simulink model "PV4x4_sweep_grp"  (R2025b)
(part 3 of 3)

  D_41_1 : ee_lib/Semiconductors & Converters/Diode  ModelType=ee.enum.diode.modelType.pwl  TableType=ee.enum.diode.tableType.IfMat  IfMat=[.07, .12, .19, 1.75, 4.24, 7.32, 11.2; .16, .3, .72, 2.14, 5.02, 8.35, 13.12] A  VfMat=[.9, 1.15, 1.25, 1.5, 1.75, 2.17, 2.6, 2.85; .58, .68, .75, 1.1, 1.38, 1.77, 2.27, 2.7] V  TjVec=[25, 125] degC  VfVec=[.5, .7, .9, 1.3, 1.7, 2.1, 2.5] V  IfVec=[.1, .2, .5, 1, 2, 4, 7, 10] A  IrMat=[1e-06, 2e-06, 5e-06, 1e-05, 2.5e-05, 5e-05, .0001; 2e-06, 5e-06, 1e-05, 4e-05, 8e-05, .0002, .0005] A  VrMat=[10, 100, 200, 250, 300, 325, 350; 10, 70, 160, 220, 270, 300, 320] V  VrVec=[10, 20, 40, 50, 70, 80, 100] V  IrVec=[1e-06, 2e-06, 5e-06, 1e-05, 2e-05, 5e-05, .0001] A  Vf=byp_Vf V  Ron=byp_Ron Ohm  Goff=byp_Goff S  prmExp=ee.enum.diode.expParam.useTwo  I12=[.0137, .545] A  V12=[.6, .7] V  RS=0 Ohm  Tmeas=298.15 K  IS=1e-12 A  ec=1  I1=0.0137 A  V1=0.6 V  N_series=1  N_parallel=1  ZenerEnable=false  Rz=0.3 Ohm  BV=inf V  C_param=ee.enum.diode.capParam.fixed  CJ=0 pF  CJ0=5 pF  Vvec=[.1, 10, 100] V  Cvec=[3.5, 1, .4] pF  VJ=1 V  Mgrad=0.5  FC=0.5  Q_param=ee.enum.diode.recoveryParam.off  iRM=-7.15 A  iF=4 A  didt=-750 A/us  trr_factor=3  trr=115 ns  Qrr=150 nA*s  Vr=-600 V  Ls=150 nH  Erec=0.03 J  TT=50 ns  tau=100 ns  T_param=ee.enum.diode.temperatureParam.off  Tdevice=298.15 K  I1_T2=0.245 A  V1_T2=0.5 V  IS_T2=1.25e-7 A  Tmeas2=125 degC  XTI_param=ee.enum.diode.xtiParam.pn  XTI=3  EG_param=ee.enum.diode.egapParam.material_si  EG=1.11 eV  dBVdT=0 V/K  enable_fault_input=simscape.enum.onoff.off  i_specify=off  i_priority=None  i=0 A  i_nominal_specify=off  i_nominal_value=1  i_nominal_unit=A  v_specify=off  v_priority=None  v=0 V  v_nominal_specify=off  v_nominal_value=1  v_nominal_unit=V  v_capacitor_specify=off  v_capacitor_priority=None  v_capacitor=0 V  v_capacitor_nominal_specify=off  v_capacitor_nominal_value=1  v_capacitor_nominal_unit=V  Qj_specify=off  Qj_priority=High  Qj=0 C  Qj_nominal_specify=off  Qj_nominal_value=1  Qj_nominal_unit=C  i_diode_specify=off  i_diode_priority=None  i_diode=0 A  i_diode_nominal_specify=off  i_diode_nominal_value=1  i_diode_nominal_unit=A  v_diode_specify=off  v_diode_priority=None  v_diode=0 V  v_diode_nominal_specify=off  v_diode_nominal_value=1  v_diode_nominal_unit=V  i_capacitor_specify=off  i_capacitor_priority=None  i_capacitor=0 A  i_capacitor_nominal_specify=off  i_capacitor_nominal_value=1  i_capacitor_nominal_unit=A  power_dissipated_specify=off  power_dissipated_priority=None  power_dissipated=0 W  power_dissipated_nominal_specify=off  power_dissipated_nominal_value=1  power_dissipated_nominal_unit=W  fidelity_level=ee.enum.diode.fidelity.includeChargeDyn  rec_loss_model=ee.enum.diode.reverseRecoveryModel.fixed  ErecVal=0 J  scaleWithIandV=true  ErecMat=zeros(2, 3) J  TjrecVec=[298.15, 398.15] K  IfrecVec=[.1, 1, 10] A  IrecVal=10 A  VrecVal=10 V  tFilter=1 / 1000 / 100 s  thermal_network_parameterization=ee.enum.thermalNetworkTopology.junctionCase  Rth=[0, 10] K/W  Rth_Cauer=[1, 3, 10] K/W  Rth_Foster=[.08, .14, .22, .16] K/W  thermal_mass_parameterization=ee.enum.thermalNetwork.timeconstant  thermal_mass=[0, 1] J/K  thermal_mass_Cauer=[.1, .3, 1] J/K  thermal_mass_Foster=[.001, .005, .05, .5] J/K  thermal_time_constant=[0, 10] s  thermal_time_constant_Cauer=[1, 3, 10] s  thermal_time_constant_Foster=[7e-05, .0007, .01, .08] s  thermal_mass_initial_temperatures=[25, 25] degC  thermal_mass_initial_temperatures_Cauer=[25, 25, 25] degC  junction_thermal_mass=0.01 J/K  Tvec_initial_Foster=[25, 25, 25, 25] degC  no_thermal_network=0  junction_temperature_specify=off  junction_temperature_priority=None  junction_temperature=25 degC  junction_temperature_nominal_specify=off  junction_temperature_nominal_value=1  junction_temperature_nominal_unit=degC
  D_41_2 : ee_lib/Semiconductors & Converters/Diode  ModelType=ee.enum.diode.modelType.pwl  TableType=ee.enum.diode.tableType.IfMat  IfMat=[.07, .12, .19, 1.75, 4.24, 7.32, 11.2; .16, .3, .72, 2.14, 5.02, 8.35, 13.12] A  VfMat=[.9, 1.15, 1.25, 1.5, 1.75, 2.17, 2.6, 2.85; .58, .68, .75, 1.1, 1.38, 1.77, 2.27, 2.7] V  TjVec=[25, 125] degC  VfVec=[.5, .7, .9, 1.3, 1.7, 2.1, 2.5] V  IfVec=[.1, .2, .5, 1, 2, 4, 7, 10] A  IrMat=[1e-06, 2e-06, 5e-06, 1e-05, 2.5e-05, 5e-05, .0001; 2e-06, 5e-06, 1e-05, 4e-05, 8e-05, .0002, .0005] A  VrMat=[10, 100, 200, 250, 300, 325, 350; 10, 70, 160, 220, 270, 300, 320] V  VrVec=[10, 20, 40, 50, 70, 80, 100] V  IrVec=[1e-06, 2e-06, 5e-06, 1e-05, 2e-05, 5e-05, .0001] A  Vf=byp_Vf V  Ron=byp_Ron Ohm  Goff=byp_Goff S  prmExp=ee.enum.diode.expParam.useTwo  I12=[.0137, .545] A  V12=[.6, .7] V  RS=0 Ohm  Tmeas=298.15 K  IS=1e-12 A  ec=1  I1=0.0137 A  V1=0.6 V  N_series=1  N_parallel=1  ZenerEnable=false  Rz=0.3 Ohm  BV=inf V  C_param=ee.enum.diode.capParam.fixed  CJ=0 pF  CJ0=5 pF  Vvec=[.1, 10, 100] V  Cvec=[3.5, 1, .4] pF  VJ=1 V  Mgrad=0.5  FC=0.5  Q_param=ee.enum.diode.recoveryParam.off  iRM=-7.15 A  iF=4 A  didt=-750 A/us  trr_factor=3  trr=115 ns  Qrr=150 nA*s  Vr=-600 V  Ls=150 nH  Erec=0.03 J  TT=50 ns  tau=100 ns  T_param=ee.enum.diode.temperatureParam.off  Tdevice=298.15 K  I1_T2=0.245 A  V1_T2=0.5 V  IS_T2=1.25e-7 A  Tmeas2=125 degC  XTI_param=ee.enum.diode.xtiParam.pn  XTI=3  EG_param=ee.enum.diode.egapParam.material_si  EG=1.11 eV  dBVdT=0 V/K  enable_fault_input=simscape.enum.onoff.off  i_specify=off  i_priority=None  i=0 A  i_nominal_specify=off  i_nominal_value=1  i_nominal_unit=A  v_specify=off  v_priority=None  v=0 V  v_nominal_specify=off  v_nominal_value=1  v_nominal_unit=V  v_capacitor_specify=off  v_capacitor_priority=None  v_capacitor=0 V  v_capacitor_nominal_specify=off  v_capacitor_nominal_value=1  v_capacitor_nominal_unit=V  Qj_specify=off  Qj_priority=High  Qj=0 C  Qj_nominal_specify=off  Qj_nominal_value=1  Qj_nominal_unit=C  i_diode_specify=off  i_diode_priority=None  i_diode=0 A  i_diode_nominal_specify=off  i_diode_nominal_value=1  i_diode_nominal_unit=A  v_diode_specify=off  v_diode_priority=None  v_diode=0 V  v_diode_nominal_specify=off  v_diode_nominal_value=1  v_diode_nominal_unit=V  i_capacitor_specify=off  i_capacitor_priority=None  i_capacitor=0 A  i_capacitor_nominal_specify=off  i_capacitor_nominal_value=1  i_capacitor_nominal_unit=A  power_dissipated_specify=off  power_dissipated_priority=None  power_dissipated=0 W  power_dissipated_nominal_specify=off  power_dissipated_nominal_value=1  power_dissipated_nominal_unit=W  fidelity_level=ee.enum.diode.fidelity.includeChargeDyn  rec_loss_model=ee.enum.diode.reverseRecoveryModel.fixed  ErecVal=0 J  scaleWithIandV=true  ErecMat=zeros(2, 3) J  TjrecVec=[298.15, 398.15] K  IfrecVec=[.1, 1, 10] A  IrecVal=10 A  VrecVal=10 V  tFilter=1 / 1000 / 100 s  thermal_network_parameterization=ee.enum.thermalNetworkTopology.junctionCase  Rth=[0, 10] K/W  Rth_Cauer=[1, 3, 10] K/W  Rth_Foster=[.08, .14, .22, .16] K/W  thermal_mass_parameterization=ee.enum.thermalNetwork.timeconstant  thermal_mass=[0, 1] J/K  thermal_mass_Cauer=[.1, .3, 1] J/K  thermal_mass_Foster=[.001, .005, .05, .5] J/K  thermal_time_constant=[0, 10] s  thermal_time_constant_Cauer=[1, 3, 10] s  thermal_time_constant_Foster=[7e-05, .0007, .01, .08] s  thermal_mass_initial_temperatures=[25, 25] degC  thermal_mass_initial_temperatures_Cauer=[25, 25, 25] degC  junction_thermal_mass=0.01 J/K  Tvec_initial_Foster=[25, 25, 25, 25] degC  no_thermal_network=0  junction_temperature_specify=off  junction_temperature_priority=None  junction_temperature=25 degC  junction_temperature_nominal_specify=off  junction_temperature_nominal_value=1  junction_temperature_nominal_unit=degC
  D_41_3 : ee_lib/Semiconductors & Converters/Diode  ModelType=ee.enum.diode.modelType.pwl  TableType=ee.enum.diode.tableType.IfMat  IfMat=[.07, .12, .19, 1.75, 4.24, 7.32, 11.2; .16, .3, .72, 2.14, 5.02, 8.35, 13.12] A  VfMat=[.9, 1.15, 1.25, 1.5, 1.75, 2.17, 2.6, 2.85; .58, .68, .75, 1.1, 1.38, 1.77, 2.27, 2.7] V  TjVec=[25, 125] degC  VfVec=[.5, .7, .9, 1.3, 1.7, 2.1, 2.5] V  IfVec=[.1, .2, .5, 1, 2, 4, 7, 10] A  IrMat=[1e-06, 2e-06, 5e-06, 1e-05, 2.5e-05, 5e-05, .0001; 2e-06, 5e-06, 1e-05, 4e-05, 8e-05, .0002, .0005] A  VrMat=[10, 100, 200, 250, 300, 325, 350; 10, 70, 160, 220, 270, 300, 320] V  VrVec=[10, 20, 40, 50, 70, 80, 100] V  IrVec=[1e-06, 2e-06, 5e-06, 1e-05, 2e-05, 5e-05, .0001] A  Vf=byp_Vf V  Ron=byp_Ron Ohm  Goff=byp_Goff S  prmExp=ee.enum.diode.expParam.useTwo  I12=[.0137, .545] A  V12=[.6, .7] V  RS=0 Ohm  Tmeas=298.15 K  IS=1e-12 A  ec=1  I1=0.0137 A  V1=0.6 V  N_series=1  N_parallel=1  ZenerEnable=false  Rz=0.3 Ohm  BV=inf V  C_param=ee.enum.diode.capParam.fixed  CJ=0 pF  CJ0=5 pF  Vvec=[.1, 10, 100] V  Cvec=[3.5, 1, .4] pF  VJ=1 V  Mgrad=0.5  FC=0.5  Q_param=ee.enum.diode.recoveryParam.off  iRM=-7.15 A  iF=4 A  didt=-750 A/us  trr_factor=3  trr=115 ns  Qrr=150 nA*s  Vr=-600 V  Ls=150 nH  Erec=0.03 J  TT=50 ns  tau=100 ns  T_param=ee.enum.diode.temperatureParam.off  Tdevice=298.15 K  I1_T2=0.245 A  V1_T2=0.5 V  IS_T2=1.25e-7 A  Tmeas2=125 degC  XTI_param=ee.enum.diode.xtiParam.pn  XTI=3  EG_param=ee.enum.diode.egapParam.material_si  EG=1.11 eV  dBVdT=0 V/K  enable_fault_input=simscape.enum.onoff.off  i_specify=off  i_priority=None  i=0 A  i_nominal_specify=off  i_nominal_value=1  i_nominal_unit=A  v_specify=off  v_priority=None  v=0 V  v_nominal_specify=off  v_nominal_value=1  v_nominal_unit=V  v_capacitor_specify=off  v_capacitor_priority=None  v_capacitor=0 V  v_capacitor_nominal_specify=off  v_capacitor_nominal_value=1  v_capacitor_nominal_unit=V  Qj_specify=off  Qj_priority=High  Qj=0 C  Qj_nominal_specify=off  Qj_nominal_value=1  Qj_nominal_unit=C  i_diode_specify=off  i_diode_priority=None  i_diode=0 A  i_diode_nominal_specify=off  i_diode_nominal_value=1  i_diode_nominal_unit=A  v_diode_specify=off  v_diode_priority=None  v_diode=0 V  v_diode_nominal_specify=off  v_diode_nominal_value=1  v_diode_nominal_unit=V  i_capacitor_specify=off  i_capacitor_priority=None  i_capacitor=0 A  i_capacitor_nominal_specify=off  i_capacitor_nominal_value=1  i_capacitor_nominal_unit=A  power_dissipated_specify=off  power_dissipated_priority=None  power_dissipated=0 W  power_dissipated_nominal_specify=off  power_dissipated_nominal_value=1  power_dissipated_nominal_unit=W  fidelity_level=ee.enum.diode.fidelity.includeChargeDyn  rec_loss_model=ee.enum.diode.reverseRecoveryModel.fixed  ErecVal=0 J  scaleWithIandV=true  ErecMat=zeros(2, 3) J  TjrecVec=[298.15, 398.15] K  IfrecVec=[.1, 1, 10] A  IrecVal=10 A  VrecVal=10 V  tFilter=1 / 1000 / 100 s  thermal_network_parameterization=ee.enum.thermalNetworkTopology.junctionCase  Rth=[0, 10] K/W  Rth_Cauer=[1, 3, 10] K/W  Rth_Foster=[.08, .14, .22, .16] K/W  thermal_mass_parameterization=ee.enum.thermalNetwork.timeconstant  thermal_mass=[0, 1] J/K  thermal_mass_Cauer=[.1, .3, 1] J/K  thermal_mass_Foster=[.001, .005, .05, .5] J/K  thermal_time_constant=[0, 10] s  thermal_time_constant_Cauer=[1, 3, 10] s  thermal_time_constant_Foster=[7e-05, .0007, .01, .08] s  thermal_mass_initial_temperatures=[25, 25] degC  thermal_mass_initial_temperatures_Cauer=[25, 25, 25] degC  junction_thermal_mass=0.01 J/K  Tvec_initial_Foster=[25, 25, 25, 25] degC  no_thermal_network=0  junction_temperature_specify=off  junction_temperature_priority=None  junction_temperature=25 degC  junction_temperature_nominal_specify=off  junction_temperature_nominal_value=1  junction_temperature_nominal_unit=degC
  D_42_1 : ee_lib/Semiconductors & Converters/Diode  ModelType=ee.enum.diode.modelType.pwl  TableType=ee.enum.diode.tableType.IfMat  IfMat=[.07, .12, .19, 1.75, 4.24, 7.32, 11.2; .16, .3, .72, 2.14, 5.02, 8.35, 13.12] A  VfMat=[.9, 1.15, 1.25, 1.5, 1.75, 2.17, 2.6, 2.85; .58, .68, .75, 1.1, 1.38, 1.77, 2.27, 2.7] V  TjVec=[25, 125] degC  VfVec=[.5, .7, .9, 1.3, 1.7, 2.1, 2.5] V  IfVec=[.1, .2, .5, 1, 2, 4, 7, 10] A  IrMat=[1e-06, 2e-06, 5e-06, 1e-05, 2.5e-05, 5e-05, .0001; 2e-06, 5e-06, 1e-05, 4e-05, 8e-05, .0002, .0005] A  VrMat=[10, 100, 200, 250, 300, 325, 350; 10, 70, 160, 220, 270, 300, 320] V  VrVec=[10, 20, 40, 50, 70, 80, 100] V  IrVec=[1e-06, 2e-06, 5e-06, 1e-05, 2e-05, 5e-05, .0001] A  Vf=byp_Vf V  Ron=byp_Ron Ohm  Goff=byp_Goff S  prmExp=ee.enum.diode.expParam.useTwo  I12=[.0137, .545] A  V12=[.6, .7] V  RS=0 Ohm  Tmeas=298.15 K  IS=1e-12 A  ec=1  I1=0.0137 A  V1=0.6 V  N_series=1  N_parallel=1  ZenerEnable=false  Rz=0.3 Ohm  BV=inf V  C_param=ee.enum.diode.capParam.fixed  CJ=0 pF  CJ0=5 pF  Vvec=[.1, 10, 100] V  Cvec=[3.5, 1, .4] pF  VJ=1 V  Mgrad=0.5  FC=0.5  Q_param=ee.enum.diode.recoveryParam.off  iRM=-7.15 A  iF=4 A  didt=-750 A/us  trr_factor=3  trr=115 ns  Qrr=150 nA*s  Vr=-600 V  Ls=150 nH  Erec=0.03 J  TT=50 ns  tau=100 ns  T_param=ee.enum.diode.temperatureParam.off  Tdevice=298.15 K  I1_T2=0.245 A  V1_T2=0.5 V  IS_T2=1.25e-7 A  Tmeas2=125 degC  XTI_param=ee.enum.diode.xtiParam.pn  XTI=3  EG_param=ee.enum.diode.egapParam.material_si  EG=1.11 eV  dBVdT=0 V/K  enable_fault_input=simscape.enum.onoff.off  i_specify=off  i_priority=None  i=0 A  i_nominal_specify=off  i_nominal_value=1  i_nominal_unit=A  v_specify=off  v_priority=None  v=0 V  v_nominal_specify=off  v_nominal_value=1  v_nominal_unit=V  v_capacitor_specify=off  v_capacitor_priority=None  v_capacitor=0 V  v_capacitor_nominal_specify=off  v_capacitor_nominal_value=1  v_capacitor_nominal_unit=V  Qj_specify=off  Qj_priority=High  Qj=0 C  Qj_nominal_specify=off  Qj_nominal_value=1  Qj_nominal_unit=C  i_diode_specify=off  i_diode_priority=None  i_diode=0 A  i_diode_nominal_specify=off  i_diode_nominal_value=1  i_diode_nominal_unit=A  v_diode_specify=off  v_diode_priority=None  v_diode=0 V  v_diode_nominal_specify=off  v_diode_nominal_value=1  v_diode_nominal_unit=V  i_capacitor_specify=off  i_capacitor_priority=None  i_capacitor=0 A  i_capacitor_nominal_specify=off  i_capacitor_nominal_value=1  i_capacitor_nominal_unit=A  power_dissipated_specify=off  power_dissipated_priority=None  power_dissipated=0 W  power_dissipated_nominal_specify=off  power_dissipated_nominal_value=1  power_dissipated_nominal_unit=W  fidelity_level=ee.enum.diode.fidelity.includeChargeDyn  rec_loss_model=ee.enum.diode.reverseRecoveryModel.fixed  ErecVal=0 J  scaleWithIandV=true  ErecMat=zeros(2, 3) J  TjrecVec=[298.15, 398.15] K  IfrecVec=[.1, 1, 10] A  IrecVal=10 A  VrecVal=10 V  tFilter=1 / 1000 / 100 s  thermal_network_parameterization=ee.enum.thermalNetworkTopology.junctionCase  Rth=[0, 10] K/W  Rth_Cauer=[1, 3, 10] K/W  Rth_Foster=[.08, .14, .22, .16] K/W  thermal_mass_parameterization=ee.enum.thermalNetwork.timeconstant  thermal_mass=[0, 1] J/K  thermal_mass_Cauer=[.1, .3, 1] J/K  thermal_mass_Foster=[.001, .005, .05, .5] J/K  thermal_time_constant=[0, 10] s  thermal_time_constant_Cauer=[1, 3, 10] s  thermal_time_constant_Foster=[7e-05, .0007, .01, .08] s  thermal_mass_initial_temperatures=[25, 25] degC  thermal_mass_initial_temperatures_Cauer=[25, 25, 25] degC  junction_thermal_mass=0.01 J/K  Tvec_initial_Foster=[25, 25, 25, 25] degC  no_thermal_network=0  junction_temperature_specify=off  junction_temperature_priority=None  junction_temperature=25 degC  junction_temperature_nominal_specify=off  junction_temperature_nominal_value=1  junction_temperature_nominal_unit=degC
  D_42_2 : ee_lib/Semiconductors & Converters/Diode  ModelType=ee.enum.diode.modelType.pwl  TableType=ee.enum.diode.tableType.IfMat  IfMat=[.07, .12, .19, 1.75, 4.24, 7.32, 11.2; .16, .3, .72, 2.14, 5.02, 8.35, 13.12] A  VfMat=[.9, 1.15, 1.25, 1.5, 1.75, 2.17, 2.6, 2.85; .58, .68, .75, 1.1, 1.38, 1.77, 2.27, 2.7] V  TjVec=[25, 125] degC  VfVec=[.5, .7, .9, 1.3, 1.7, 2.1, 2.5] V  IfVec=[.1, .2, .5, 1, 2, 4, 7, 10] A  IrMat=[1e-06, 2e-06, 5e-06, 1e-05, 2.5e-05, 5e-05, .0001; 2e-06, 5e-06, 1e-05, 4e-05, 8e-05, .0002, .0005] A  VrMat=[10, 100, 200, 250, 300, 325, 350; 10, 70, 160, 220, 270, 300, 320] V  VrVec=[10, 20, 40, 50, 70, 80, 100] V  IrVec=[1e-06, 2e-06, 5e-06, 1e-05, 2e-05, 5e-05, .0001] A  Vf=byp_Vf V  Ron=byp_Ron Ohm  Goff=byp_Goff S  prmExp=ee.enum.diode.expParam.useTwo  I12=[.0137, .545] A  V12=[.6, .7] V  RS=0 Ohm  Tmeas=298.15 K  IS=1e-12 A  ec=1  I1=0.0137 A  V1=0.6 V  N_series=1  N_parallel=1  ZenerEnable=false  Rz=0.3 Ohm  BV=inf V  C_param=ee.enum.diode.capParam.fixed  CJ=0 pF  CJ0=5 pF  Vvec=[.1, 10, 100] V  Cvec=[3.5, 1, .4] pF  VJ=1 V  Mgrad=0.5  FC=0.5  Q_param=ee.enum.diode.recoveryParam.off  iRM=-7.15 A  iF=4 A  didt=-750 A/us  trr_factor=3  trr=115 ns  Qrr=150 nA*s  Vr=-600 V  Ls=150 nH  Erec=0.03 J  TT=50 ns  tau=100 ns  T_param=ee.enum.diode.temperatureParam.off  Tdevice=298.15 K  I1_T2=0.245 A  V1_T2=0.5 V  IS_T2=1.25e-7 A  Tmeas2=125 degC  XTI_param=ee.enum.diode.xtiParam.pn  XTI=3  EG_param=ee.enum.diode.egapParam.material_si  EG=1.11 eV  dBVdT=0 V/K  enable_fault_input=simscape.enum.onoff.off  i_specify=off  i_priority=None  i=0 A  i_nominal_specify=off  i_nominal_value=1  i_nominal_unit=A  v_specify=off  v_priority=None  v=0 V  v_nominal_specify=off  v_nominal_value=1  v_nominal_unit=V  v_capacitor_specify=off  v_capacitor_priority=None  v_capacitor=0 V  v_capacitor_nominal_specify=off  v_capacitor_nominal_value=1  v_capacitor_nominal_unit=V  Qj_specify=off  Qj_priority=High  Qj=0 C  Qj_nominal_specify=off  Qj_nominal_value=1  Qj_nominal_unit=C  i_diode_specify=off  i_diode_priority=None  i_diode=0 A  i_diode_nominal_specify=off  i_diode_nominal_value=1  i_diode_nominal_unit=A  v_diode_specify=off  v_diode_priority=None  v_diode=0 V  v_diode_nominal_specify=off  v_diode_nominal_value=1  v_diode_nominal_unit=V  i_capacitor_specify=off  i_capacitor_priority=None  i_capacitor=0 A  i_capacitor_nominal_specify=off  i_capacitor_nominal_value=1  i_capacitor_nominal_unit=A  power_dissipated_specify=off  power_dissipated_priority=None  power_dissipated=0 W  power_dissipated_nominal_specify=off  power_dissipated_nominal_value=1  power_dissipated_nominal_unit=W  fidelity_level=ee.enum.diode.fidelity.includeChargeDyn  rec_loss_model=ee.enum.diode.reverseRecoveryModel.fixed  ErecVal=0 J  scaleWithIandV=true  ErecMat=zeros(2, 3) J  TjrecVec=[298.15, 398.15] K  IfrecVec=[.1, 1, 10] A  IrecVal=10 A  VrecVal=10 V  tFilter=1 / 1000 / 100 s  thermal_network_parameterization=ee.enum.thermalNetworkTopology.junctionCase  Rth=[0, 10] K/W  Rth_Cauer=[1, 3, 10] K/W  Rth_Foster=[.08, .14, .22, .16] K/W  thermal_mass_parameterization=ee.enum.thermalNetwork.timeconstant  thermal_mass=[0, 1] J/K  thermal_mass_Cauer=[.1, .3, 1] J/K  thermal_mass_Foster=[.001, .005, .05, .5] J/K  thermal_time_constant=[0, 10] s  thermal_time_constant_Cauer=[1, 3, 10] s  thermal_time_constant_Foster=[7e-05, .0007, .01, .08] s  thermal_mass_initial_temperatures=[25, 25] degC  thermal_mass_initial_temperatures_Cauer=[25, 25, 25] degC  junction_thermal_mass=0.01 J/K  Tvec_initial_Foster=[25, 25, 25, 25] degC  no_thermal_network=0  junction_temperature_specify=off  junction_temperature_priority=None  junction_temperature=25 degC  junction_temperature_nominal_specify=off  junction_temperature_nominal_value=1  junction_temperature_nominal_unit=degC
  D_42_3 : ee_lib/Semiconductors & Converters/Diode  ModelType=ee.enum.diode.modelType.pwl  TableType=ee.enum.diode.tableType.IfMat  IfMat=[.07, .12, .19, 1.75, 4.24, 7.32, 11.2; .16, .3, .72, 2.14, 5.02, 8.35, 13.12] A  VfMat=[.9, 1.15, 1.25, 1.5, 1.75, 2.17, 2.6, 2.85; .58, .68, .75, 1.1, 1.38, 1.77, 2.27, 2.7] V  TjVec=[25, 125] degC  VfVec=[.5, .7, .9, 1.3, 1.7, 2.1, 2.5] V  IfVec=[.1, .2, .5, 1, 2, 4, 7, 10] A  IrMat=[1e-06, 2e-06, 5e-06, 1e-05, 2.5e-05, 5e-05, .0001; 2e-06, 5e-06, 1e-05, 4e-05, 8e-05, .0002, .0005] A  VrMat=[10, 100, 200, 250, 300, 325, 350; 10, 70, 160, 220, 270, 300, 320] V  VrVec=[10, 20, 40, 50, 70, 80, 100] V  IrVec=[1e-06, 2e-06, 5e-06, 1e-05, 2e-05, 5e-05, .0001] A  Vf=byp_Vf V  Ron=byp_Ron Ohm  Goff=byp_Goff S  prmExp=ee.enum.diode.expParam.useTwo  I12=[.0137, .545] A  V12=[.6, .7] V  RS=0 Ohm  Tmeas=298.15 K  IS=1e-12 A  ec=1  I1=0.0137 A  V1=0.6 V  N_series=1  N_parallel=1  ZenerEnable=false  Rz=0.3 Ohm  BV=inf V  C_param=ee.enum.diode.capParam.fixed  CJ=0 pF  CJ0=5 pF  Vvec=[.1, 10, 100] V  Cvec=[3.5, 1, .4] pF  VJ=1 V  Mgrad=0.5  FC=0.5  Q_param=ee.enum.diode.recoveryParam.off  iRM=-7.15 A  iF=4 A  didt=-750 A/us  trr_factor=3  trr=115 ns  Qrr=150 nA*s  Vr=-600 V  Ls=150 nH  Erec=0.03 J  TT=50 ns  tau=100 ns  T_param=ee.enum.diode.temperatureParam.off  Tdevice=298.15 K  I1_T2=0.245 A  V1_T2=0.5 V  IS_T2=1.25e-7 A  Tmeas2=125 degC  XTI_param=ee.enum.diode.xtiParam.pn  XTI=3  EG_param=ee.enum.diode.egapParam.material_si  EG=1.11 eV  dBVdT=0 V/K  enable_fault_input=simscape.enum.onoff.off  i_specify=off  i_priority=None  i=0 A  i_nominal_specify=off  i_nominal_value=1  i_nominal_unit=A  v_specify=off  v_priority=None  v=0 V  v_nominal_specify=off  v_nominal_value=1  v_nominal_unit=V  v_capacitor_specify=off  v_capacitor_priority=None  v_capacitor=0 V  v_capacitor_nominal_specify=off  v_capacitor_nominal_value=1  v_capacitor_nominal_unit=V  Qj_specify=off  Qj_priority=High  Qj=0 C  Qj_nominal_specify=off  Qj_nominal_value=1  Qj_nominal_unit=C  i_diode_specify=off  i_diode_priority=None  i_diode=0 A  i_diode_nominal_specify=off  i_diode_nominal_value=1  i_diode_nominal_unit=A  v_diode_specify=off  v_diode_priority=None  v_diode=0 V  v_diode_nominal_specify=off  v_diode_nominal_value=1  v_diode_nominal_unit=V  i_capacitor_specify=off  i_capacitor_priority=None  i_capacitor=0 A  i_capacitor_nominal_specify=off  i_capacitor_nominal_value=1  i_capacitor_nominal_unit=A  power_dissipated_specify=off  power_dissipated_priority=None  power_dissipated=0 W  power_dissipated_nominal_specify=off  power_dissipated_nominal_value=1  power_dissipated_nominal_unit=W  fidelity_level=ee.enum.diode.fidelity.includeChargeDyn  rec_loss_model=ee.enum.diode.reverseRecoveryModel.fixed  ErecVal=0 J  scaleWithIandV=true  ErecMat=zeros(2, 3) J  TjrecVec=[298.15, 398.15] K  IfrecVec=[.1, 1, 10] A  IrecVal=10 A  VrecVal=10 V  tFilter=1 / 1000 / 100 s  thermal_network_parameterization=ee.enum.thermalNetworkTopology.junctionCase  Rth=[0, 10] K/W  Rth_Cauer=[1, 3, 10] K/W  Rth_Foster=[.08, .14, .22, .16] K/W  thermal_mass_parameterization=ee.enum.thermalNetwork.timeconstant  thermal_mass=[0, 1] J/K  thermal_mass_Cauer=[.1, .3, 1] J/K  thermal_mass_Foster=[.001, .005, .05, .5] J/K  thermal_time_constant=[0, 10] s  thermal_time_constant_Cauer=[1, 3, 10] s  thermal_time_constant_Foster=[7e-05, .0007, .01, .08] s  thermal_mass_initial_temperatures=[25, 25] degC  thermal_mass_initial_temperatures_Cauer=[25, 25, 25] degC  junction_thermal_mass=0.01 J/K  Tvec_initial_Foster=[25, 25, 25, 25] degC  no_thermal_network=0  junction_temperature_specify=off  junction_temperature_priority=None  junction_temperature=25 degC  junction_temperature_nominal_specify=off  junction_temperature_nominal_value=1  junction_temperature_nominal_unit=degC
  D_43_1 : ee_lib/Semiconductors & Converters/Diode  ModelType=ee.enum.diode.modelType.pwl  TableType=ee.enum.diode.tableType.IfMat  IfMat=[.07, .12, .19, 1.75, 4.24, 7.32, 11.2; .16, .3, .72, 2.14, 5.02, 8.35, 13.12] A  VfMat=[.9, 1.15, 1.25, 1.5, 1.75, 2.17, 2.6, 2.85; .58, .68, .75, 1.1, 1.38, 1.77, 2.27, 2.7] V  TjVec=[25, 125] degC  VfVec=[.5, .7, .9, 1.3, 1.7, 2.1, 2.5] V  IfVec=[.1, .2, .5, 1, 2, 4, 7, 10] A  IrMat=[1e-06, 2e-06, 5e-06, 1e-05, 2.5e-05, 5e-05, .0001; 2e-06, 5e-06, 1e-05, 4e-05, 8e-05, .0002, .0005] A  VrMat=[10, 100, 200, 250, 300, 325, 350; 10, 70, 160, 220, 270, 300, 320] V  VrVec=[10, 20, 40, 50, 70, 80, 100] V  IrVec=[1e-06, 2e-06, 5e-06, 1e-05, 2e-05, 5e-05, .0001] A  Vf=byp_Vf V  Ron=byp_Ron Ohm  Goff=byp_Goff S  prmExp=ee.enum.diode.expParam.useTwo  I12=[.0137, .545] A  V12=[.6, .7] V  RS=0 Ohm  Tmeas=298.15 K  IS=1e-12 A  ec=1  I1=0.0137 A  V1=0.6 V  N_series=1  N_parallel=1  ZenerEnable=false  Rz=0.3 Ohm  BV=inf V  C_param=ee.enum.diode.capParam.fixed  CJ=0 pF  CJ0=5 pF  Vvec=[.1, 10, 100] V  Cvec=[3.5, 1, .4] pF  VJ=1 V  Mgrad=0.5  FC=0.5  Q_param=ee.enum.diode.recoveryParam.off  iRM=-7.15 A  iF=4 A  didt=-750 A/us  trr_factor=3  trr=115 ns  Qrr=150 nA*s  Vr=-600 V  Ls=150 nH  Erec=0.03 J  TT=50 ns  tau=100 ns  T_param=ee.enum.diode.temperatureParam.off  Tdevice=298.15 K  I1_T2=0.245 A  V1_T2=0.5 V  IS_T2=1.25e-7 A  Tmeas2=125 degC  XTI_param=ee.enum.diode.xtiParam.pn  XTI=3  EG_param=ee.enum.diode.egapParam.material_si  EG=1.11 eV  dBVdT=0 V/K  enable_fault_input=simscape.enum.onoff.off  i_specify=off  i_priority=None  i=0 A  i_nominal_specify=off  i_nominal_value=1  i_nominal_unit=A  v_specify=off  v_priority=None  v=0 V  v_nominal_specify=off  v_nominal_value=1  v_nominal_unit=V  v_capacitor_specify=off  v_capacitor_priority=None  v_capacitor=0 V  v_capacitor_nominal_specify=off  v_capacitor_nominal_value=1  v_capacitor_nominal_unit=V  Qj_specify=off  Qj_priority=High  Qj=0 C  Qj_nominal_specify=off  Qj_nominal_value=1  Qj_nominal_unit=C  i_diode_specify=off  i_diode_priority=None  i_diode=0 A  i_diode_nominal_specify=off  i_diode_nominal_value=1  i_diode_nominal_unit=A  v_diode_specify=off  v_diode_priority=None  v_diode=0 V  v_diode_nominal_specify=off  v_diode_nominal_value=1  v_diode_nominal_unit=V  i_capacitor_specify=off  i_capacitor_priority=None  i_capacitor=0 A  i_capacitor_nominal_specify=off  i_capacitor_nominal_value=1  i_capacitor_nominal_unit=A  power_dissipated_specify=off  power_dissipated_priority=None  power_dissipated=0 W  power_dissipated_nominal_specify=off  power_dissipated_nominal_value=1  power_dissipated_nominal_unit=W  fidelity_level=ee.enum.diode.fidelity.includeChargeDyn  rec_loss_model=ee.enum.diode.reverseRecoveryModel.fixed  ErecVal=0 J  scaleWithIandV=true  ErecMat=zeros(2, 3) J  TjrecVec=[298.15, 398.15] K  IfrecVec=[.1, 1, 10] A  IrecVal=10 A  VrecVal=10 V  tFilter=1 / 1000 / 100 s  thermal_network_parameterization=ee.enum.thermalNetworkTopology.junctionCase  Rth=[0, 10] K/W  Rth_Cauer=[1, 3, 10] K/W  Rth_Foster=[.08, .14, .22, .16] K/W  thermal_mass_parameterization=ee.enum.thermalNetwork.timeconstant  thermal_mass=[0, 1] J/K  thermal_mass_Cauer=[.1, .3, 1] J/K  thermal_mass_Foster=[.001, .005, .05, .5] J/K  thermal_time_constant=[0, 10] s  thermal_time_constant_Cauer=[1, 3, 10] s  thermal_time_constant_Foster=[7e-05, .0007, .01, .08] s  thermal_mass_initial_temperatures=[25, 25] degC  thermal_mass_initial_temperatures_Cauer=[25, 25, 25] degC  junction_thermal_mass=0.01 J/K  Tvec_initial_Foster=[25, 25, 25, 25] degC  no_thermal_network=0  junction_temperature_specify=off  junction_temperature_priority=None  junction_temperature=25 degC  junction_temperature_nominal_specify=off  junction_temperature_nominal_value=1  junction_temperature_nominal_unit=degC
  D_43_2 : ee_lib/Semiconductors & Converters/Diode  ModelType=ee.enum.diode.modelType.pwl  TableType=ee.enum.diode.tableType.IfMat  IfMat=[.07, .12, .19, 1.75, 4.24, 7.32, 11.2; .16, .3, .72, 2.14, 5.02, 8.35, 13.12] A  VfMat=[.9, 1.15, 1.25, 1.5, 1.75, 2.17, 2.6, 2.85; .58, .68, .75, 1.1, 1.38, 1.77, 2.27, 2.7] V  TjVec=[25, 125] degC  VfVec=[.5, .7, .9, 1.3, 1.7, 2.1, 2.5] V  IfVec=[.1, .2, .5, 1, 2, 4, 7, 10] A  IrMat=[1e-06, 2e-06, 5e-06, 1e-05, 2.5e-05, 5e-05, .0001; 2e-06, 5e-06, 1e-05, 4e-05, 8e-05, .0002, .0005] A  VrMat=[10, 100, 200, 250, 300, 325, 350; 10, 70, 160, 220, 270, 300, 320] V  VrVec=[10, 20, 40, 50, 70, 80, 100] V  IrVec=[1e-06, 2e-06, 5e-06, 1e-05, 2e-05, 5e-05, .0001] A  Vf=byp_Vf V  Ron=byp_Ron Ohm  Goff=byp_Goff S  prmExp=ee.enum.diode.expParam.useTwo  I12=[.0137, .545] A  V12=[.6, .7] V  RS=0 Ohm  Tmeas=298.15 K  IS=1e-12 A  ec=1  I1=0.0137 A  V1=0.6 V  N_series=1  N_parallel=1  ZenerEnable=false  Rz=0.3 Ohm  BV=inf V  C_param=ee.enum.diode.capParam.fixed  CJ=0 pF  CJ0=5 pF  Vvec=[.1, 10, 100] V  Cvec=[3.5, 1, .4] pF  VJ=1 V  Mgrad=0.5  FC=0.5  Q_param=ee.enum.diode.recoveryParam.off  iRM=-7.15 A  iF=4 A  didt=-750 A/us  trr_factor=3  trr=115 ns  Qrr=150 nA*s  Vr=-600 V  Ls=150 nH  Erec=0.03 J  TT=50 ns  tau=100 ns  T_param=ee.enum.diode.temperatureParam.off  Tdevice=298.15 K  I1_T2=0.245 A  V1_T2=0.5 V  IS_T2=1.25e-7 A  Tmeas2=125 degC  XTI_param=ee.enum.diode.xtiParam.pn  XTI=3  EG_param=ee.enum.diode.egapParam.material_si  EG=1.11 eV  dBVdT=0 V/K  enable_fault_input=simscape.enum.onoff.off  i_specify=off  i_priority=None  i=0 A  i_nominal_specify=off  i_nominal_value=1  i_nominal_unit=A  v_specify=off  v_priority=None  v=0 V  v_nominal_specify=off  v_nominal_value=1  v_nominal_unit=V  v_capacitor_specify=off  v_capacitor_priority=None  v_capacitor=0 V  v_capacitor_nominal_specify=off  v_capacitor_nominal_value=1  v_capacitor_nominal_unit=V  Qj_specify=off  Qj_priority=High  Qj=0 C  Qj_nominal_specify=off  Qj_nominal_value=1  Qj_nominal_unit=C  i_diode_specify=off  i_diode_priority=None  i_diode=0 A  i_diode_nominal_specify=off  i_diode_nominal_value=1  i_diode_nominal_unit=A  v_diode_specify=off  v_diode_priority=None  v_diode=0 V  v_diode_nominal_specify=off  v_diode_nominal_value=1  v_diode_nominal_unit=V  i_capacitor_specify=off  i_capacitor_priority=None  i_capacitor=0 A  i_capacitor_nominal_specify=off  i_capacitor_nominal_value=1  i_capacitor_nominal_unit=A  power_dissipated_specify=off  power_dissipated_priority=None  power_dissipated=0 W  power_dissipated_nominal_specify=off  power_dissipated_nominal_value=1  power_dissipated_nominal_unit=W  fidelity_level=ee.enum.diode.fidelity.includeChargeDyn  rec_loss_model=ee.enum.diode.reverseRecoveryModel.fixed  ErecVal=0 J  scaleWithIandV=true  ErecMat=zeros(2, 3) J  TjrecVec=[298.15, 398.15] K  IfrecVec=[.1, 1, 10] A  IrecVal=10 A  VrecVal=10 V  tFilter=1 / 1000 / 100 s  thermal_network_parameterization=ee.enum.thermalNetworkTopology.junctionCase  Rth=[0, 10] K/W  Rth_Cauer=[1, 3, 10] K/W  Rth_Foster=[.08, .14, .22, .16] K/W  thermal_mass_parameterization=ee.enum.thermalNetwork.timeconstant  thermal_mass=[0, 1] J/K  thermal_mass_Cauer=[.1, .3, 1] J/K  thermal_mass_Foster=[.001, .005, .05, .5] J/K  thermal_time_constant=[0, 10] s  thermal_time_constant_Cauer=[1, 3, 10] s  thermal_time_constant_Foster=[7e-05, .0007, .01, .08] s  thermal_mass_initial_temperatures=[25, 25] degC  thermal_mass_initial_temperatures_Cauer=[25, 25, 25] degC  junction_thermal_mass=0.01 J/K  Tvec_initial_Foster=[25, 25, 25, 25] degC  no_thermal_network=0  junction_temperature_specify=off  junction_temperature_priority=None  junction_temperature=25 degC  junction_temperature_nominal_specify=off  junction_temperature_nominal_value=1  junction_temperature_nominal_unit=degC
  D_43_3 : ee_lib/Semiconductors & Converters/Diode  ModelType=ee.enum.diode.modelType.pwl  TableType=ee.enum.diode.tableType.IfMat  IfMat=[.07, .12, .19, 1.75, 4.24, 7.32, 11.2; .16, .3, .72, 2.14, 5.02, 8.35, 13.12] A  VfMat=[.9, 1.15, 1.25, 1.5, 1.75, 2.17, 2.6, 2.85; .58, .68, .75, 1.1, 1.38, 1.77, 2.27, 2.7] V  TjVec=[25, 125] degC  VfVec=[.5, .7, .9, 1.3, 1.7, 2.1, 2.5] V  IfVec=[.1, .2, .5, 1, 2, 4, 7, 10] A  IrMat=[1e-06, 2e-06, 5e-06, 1e-05, 2.5e-05, 5e-05, .0001; 2e-06, 5e-06, 1e-05, 4e-05, 8e-05, .0002, .0005] A  VrMat=[10, 100, 200, 250, 300, 325, 350; 10, 70, 160, 220, 270, 300, 320] V  VrVec=[10, 20, 40, 50, 70, 80, 100] V  IrVec=[1e-06, 2e-06, 5e-06, 1e-05, 2e-05, 5e-05, .0001] A  Vf=byp_Vf V  Ron=byp_Ron Ohm  Goff=byp_Goff S  prmExp=ee.enum.diode.expParam.useTwo  I12=[.0137, .545] A  V12=[.6, .7] V  RS=0 Ohm  Tmeas=298.15 K  IS=1e-12 A  ec=1  I1=0.0137 A  V1=0.6 V  N_series=1  N_parallel=1  ZenerEnable=false  Rz=0.3 Ohm  BV=inf V  C_param=ee.enum.diode.capParam.fixed  CJ=0 pF  CJ0=5 pF  Vvec=[.1, 10, 100] V  Cvec=[3.5, 1, .4] pF  VJ=1 V  Mgrad=0.5  FC=0.5  Q_param=ee.enum.diode.recoveryParam.off  iRM=-7.15 A  iF=4 A  didt=-750 A/us  trr_factor=3  trr=115 ns  Qrr=150 nA*s  Vr=-600 V  Ls=150 nH  Erec=0.03 J  TT=50 ns  tau=100 ns  T_param=ee.enum.diode.temperatureParam.off  Tdevice=298.15 K  I1_T2=0.245 A  V1_T2=0.5 V  IS_T2=1.25e-7 A  Tmeas2=125 degC  XTI_param=ee.enum.diode.xtiParam.pn  XTI=3  EG_param=ee.enum.diode.egapParam.material_si  EG=1.11 eV  dBVdT=0 V/K  enable_fault_input=simscape.enum.onoff.off  i_specify=off  i_priority=None  i=0 A  i_nominal_specify=off  i_nominal_value=1  i_nominal_unit=A  v_specify=off  v_priority=None  v=0 V  v_nominal_specify=off  v_nominal_value=1  v_nominal_unit=V  v_capacitor_specify=off  v_capacitor_priority=None  v_capacitor=0 V  v_capacitor_nominal_specify=off  v_capacitor_nominal_value=1  v_capacitor_nominal_unit=V  Qj_specify=off  Qj_priority=High  Qj=0 C  Qj_nominal_specify=off  Qj_nominal_value=1  Qj_nominal_unit=C  i_diode_specify=off  i_diode_priority=None  i_diode=0 A  i_diode_nominal_specify=off  i_diode_nominal_value=1  i_diode_nominal_unit=A  v_diode_specify=off  v_diode_priority=None  v_diode=0 V  v_diode_nominal_specify=off  v_diode_nominal_value=1  v_diode_nominal_unit=V  i_capacitor_specify=off  i_capacitor_priority=None  i_capacitor=0 A  i_capacitor_nominal_specify=off  i_capacitor_nominal_value=1  i_capacitor_nominal_unit=A  power_dissipated_specify=off  power_dissipated_priority=None  power_dissipated=0 W  power_dissipated_nominal_specify=off  power_dissipated_nominal_value=1  power_dissipated_nominal_unit=W  fidelity_level=ee.enum.diode.fidelity.includeChargeDyn  rec_loss_model=ee.enum.diode.reverseRecoveryModel.fixed  ErecVal=0 J  scaleWithIandV=true  ErecMat=zeros(2, 3) J  TjrecVec=[298.15, 398.15] K  IfrecVec=[.1, 1, 10] A  IrecVal=10 A  VrecVal=10 V  tFilter=1 / 1000 / 100 s  thermal_network_parameterization=ee.enum.thermalNetworkTopology.junctionCase  Rth=[0, 10] K/W  Rth_Cauer=[1, 3, 10] K/W  Rth_Foster=[.08, .14, .22, .16] K/W  thermal_mass_parameterization=ee.enum.thermalNetwork.timeconstant  thermal_mass=[0, 1] J/K  thermal_mass_Cauer=[.1, .3, 1] J/K  thermal_mass_Foster=[.001, .005, .05, .5] J/K  thermal_time_constant=[0, 10] s  thermal_time_constant_Cauer=[1, 3, 10] s  thermal_time_constant_Foster=[7e-05, .0007, .01, .08] s  thermal_mass_initial_temperatures=[25, 25] degC  thermal_mass_initial_temperatures_Cauer=[25, 25, 25] degC  junction_thermal_mass=0.01 J/K  Tvec_initial_Foster=[25, 25, 25, 25] degC  no_thermal_network=0  junction_temperature_specify=off  junction_temperature_priority=None  junction_temperature=25 degC  junction_temperature_nominal_specify=off  junction_temperature_nominal_value=1  junction_temperature_nominal_unit=degC
  D_44_1 : ee_lib/Semiconductors & Converters/Diode  ModelType=ee.enum.diode.modelType.pwl  TableType=ee.enum.diode.tableType.IfMat  IfMat=[.07, .12, .19, 1.75, 4.24, 7.32, 11.2; .16, .3, .72, 2.14, 5.02, 8.35, 13.12] A  VfMat=[.9, 1.15, 1.25, 1.5, 1.75, 2.17, 2.6, 2.85; .58, .68, .75, 1.1, 1.38, 1.77, 2.27, 2.7] V  TjVec=[25, 125] degC  VfVec=[.5, .7, .9, 1.3, 1.7, 2.1, 2.5] V  IfVec=[.1, .2, .5, 1, 2, 4, 7, 10] A  IrMat=[1e-06, 2e-06, 5e-06, 1e-05, 2.5e-05, 5e-05, .0001; 2e-06, 5e-06, 1e-05, 4e-05, 8e-05, .0002, .0005] A  VrMat=[10, 100, 200, 250, 300, 325, 350; 10, 70, 160, 220, 270, 300, 320] V  VrVec=[10, 20, 40, 50, 70, 80, 100] V  IrVec=[1e-06, 2e-06, 5e-06, 1e-05, 2e-05, 5e-05, .0001] A  Vf=byp_Vf V  Ron=byp_Ron Ohm  Goff=byp_Goff S  prmExp=ee.enum.diode.expParam.useTwo  I12=[.0137, .545] A  V12=[.6, .7] V  RS=0 Ohm  Tmeas=298.15 K  IS=1e-12 A  ec=1  I1=0.0137 A  V1=0.6 V  N_series=1  N_parallel=1  ZenerEnable=false  Rz=0.3 Ohm  BV=inf V  C_param=ee.enum.diode.capParam.fixed  CJ=0 pF  CJ0=5 pF  Vvec=[.1, 10, 100] V  Cvec=[3.5, 1, .4] pF  VJ=1 V  Mgrad=0.5  FC=0.5  Q_param=ee.enum.diode.recoveryParam.off  iRM=-7.15 A  iF=4 A  didt=-750 A/us  trr_factor=3  trr=115 ns  Qrr=150 nA*s  Vr=-600 V  Ls=150 nH  Erec=0.03 J  TT=50 ns  tau=100 ns  T_param=ee.enum.diode.temperatureParam.off  Tdevice=298.15 K  I1_T2=0.245 A  V1_T2=0.5 V  IS_T2=1.25e-7 A  Tmeas2=125 degC  XTI_param=ee.enum.diode.xtiParam.pn  XTI=3  EG_param=ee.enum.diode.egapParam.material_si  EG=1.11 eV  dBVdT=0 V/K  enable_fault_input=simscape.enum.onoff.off  i_specify=off  i_priority=None  i=0 A  i_nominal_specify=off  i_nominal_value=1  i_nominal_unit=A  v_specify=off  v_priority=None  v=0 V  v_nominal_specify=off  v_nominal_value=1  v_nominal_unit=V  v_capacitor_specify=off  v_capacitor_priority=None  v_capacitor=0 V  v_capacitor_nominal_specify=off  v_capacitor_nominal_value=1  v_capacitor_nominal_unit=V  Qj_specify=off  Qj_priority=High  Qj=0 C  Qj_nominal_specify=off  Qj_nominal_value=1  Qj_nominal_unit=C  i_diode_specify=off  i_diode_priority=None  i_diode=0 A  i_diode_nominal_specify=off  i_diode_nominal_value=1  i_diode_nominal_unit=A  v_diode_specify=off  v_diode_priority=None  v_diode=0 V  v_diode_nominal_specify=off  v_diode_nominal_value=1  v_diode_nominal_unit=V  i_capacitor_specify=off  i_capacitor_priority=None  i_capacitor=0 A  i_capacitor_nominal_specify=off  i_capacitor_nominal_value=1  i_capacitor_nominal_unit=A  power_dissipated_specify=off  power_dissipated_priority=None  power_dissipated=0 W  power_dissipated_nominal_specify=off  power_dissipated_nominal_value=1  power_dissipated_nominal_unit=W  fidelity_level=ee.enum.diode.fidelity.includeChargeDyn  rec_loss_model=ee.enum.diode.reverseRecoveryModel.fixed  ErecVal=0 J  scaleWithIandV=true  ErecMat=zeros(2, 3) J  TjrecVec=[298.15, 398.15] K  IfrecVec=[.1, 1, 10] A  IrecVal=10 A  VrecVal=10 V  tFilter=1 / 1000 / 100 s  thermal_network_parameterization=ee.enum.thermalNetworkTopology.junctionCase  Rth=[0, 10] K/W  Rth_Cauer=[1, 3, 10] K/W  Rth_Foster=[.08, .14, .22, .16] K/W  thermal_mass_parameterization=ee.enum.thermalNetwork.timeconstant  thermal_mass=[0, 1] J/K  thermal_mass_Cauer=[.1, .3, 1] J/K  thermal_mass_Foster=[.001, .005, .05, .5] J/K  thermal_time_constant=[0, 10] s  thermal_time_constant_Cauer=[1, 3, 10] s  thermal_time_constant_Foster=[7e-05, .0007, .01, .08] s  thermal_mass_initial_temperatures=[25, 25] degC  thermal_mass_initial_temperatures_Cauer=[25, 25, 25] degC  junction_thermal_mass=0.01 J/K  Tvec_initial_Foster=[25, 25, 25, 25] degC  no_thermal_network=0  junction_temperature_specify=off  junction_temperature_priority=None  junction_temperature=25 degC  junction_temperature_nominal_specify=off  junction_temperature_nominal_value=1  junction_temperature_nominal_unit=degC
  D_44_2 : ee_lib/Semiconductors & Converters/Diode  ModelType=ee.enum.diode.modelType.pwl  TableType=ee.enum.diode.tableType.IfMat  IfMat=[.07, .12, .19, 1.75, 4.24, 7.32, 11.2; .16, .3, .72, 2.14, 5.02, 8.35, 13.12] A  VfMat=[.9, 1.15, 1.25, 1.5, 1.75, 2.17, 2.6, 2.85; .58, .68, .75, 1.1, 1.38, 1.77, 2.27, 2.7] V  TjVec=[25, 125] degC  VfVec=[.5, .7, .9, 1.3, 1.7, 2.1, 2.5] V  IfVec=[.1, .2, .5, 1, 2, 4, 7, 10] A  IrMat=[1e-06, 2e-06, 5e-06, 1e-05, 2.5e-05, 5e-05, .0001; 2e-06, 5e-06, 1e-05, 4e-05, 8e-05, .0002, .0005] A  VrMat=[10, 100, 200, 250, 300, 325, 350; 10, 70, 160, 220, 270, 300, 320] V  VrVec=[10, 20, 40, 50, 70, 80, 100] V  IrVec=[1e-06, 2e-06, 5e-06, 1e-05, 2e-05, 5e-05, .0001] A  Vf=byp_Vf V  Ron=byp_Ron Ohm  Goff=byp_Goff S  prmExp=ee.enum.diode.expParam.useTwo  I12=[.0137, .545] A  V12=[.6, .7] V  RS=0 Ohm  Tmeas=298.15 K  IS=1e-12 A  ec=1  I1=0.0137 A  V1=0.6 V  N_series=1  N_parallel=1  ZenerEnable=false  Rz=0.3 Ohm  BV=inf V  C_param=ee.enum.diode.capParam.fixed  CJ=0 pF  CJ0=5 pF  Vvec=[.1, 10, 100] V  Cvec=[3.5, 1, .4] pF  VJ=1 V  Mgrad=0.5  FC=0.5  Q_param=ee.enum.diode.recoveryParam.off  iRM=-7.15 A  iF=4 A  didt=-750 A/us  trr_factor=3  trr=115 ns  Qrr=150 nA*s  Vr=-600 V  Ls=150 nH  Erec=0.03 J  TT=50 ns  tau=100 ns  T_param=ee.enum.diode.temperatureParam.off  Tdevice=298.15 K  I1_T2=0.245 A  V1_T2=0.5 V  IS_T2=1.25e-7 A  Tmeas2=125 degC  XTI_param=ee.enum.diode.xtiParam.pn  XTI=3  EG_param=ee.enum.diode.egapParam.material_si  EG=1.11 eV  dBVdT=0 V/K  enable_fault_input=simscape.enum.onoff.off  i_specify=off  i_priority=None  i=0 A  i_nominal_specify=off  i_nominal_value=1  i_nominal_unit=A  v_specify=off  v_priority=None  v=0 V  v_nominal_specify=off  v_nominal_value=1  v_nominal_unit=V  v_capacitor_specify=off  v_capacitor_priority=None  v_capacitor=0 V  v_capacitor_nominal_specify=off  v_capacitor_nominal_value=1  v_capacitor_nominal_unit=V  Qj_specify=off  Qj_priority=High  Qj=0 C  Qj_nominal_specify=off  Qj_nominal_value=1  Qj_nominal_unit=C  i_diode_specify=off  i_diode_priority=None  i_diode=0 A  i_diode_nominal_specify=off  i_diode_nominal_value=1  i_diode_nominal_unit=A  v_diode_specify=off  v_diode_priority=None  v_diode=0 V  v_diode_nominal_specify=off  v_diode_nominal_value=1  v_diode_nominal_unit=V  i_capacitor_specify=off  i_capacitor_priority=None  i_capacitor=0 A  i_capacitor_nominal_specify=off  i_capacitor_nominal_value=1  i_capacitor_nominal_unit=A  power_dissipated_specify=off  power_dissipated_priority=None  power_dissipated=0 W  power_dissipated_nominal_specify=off  power_dissipated_nominal_value=1  power_dissipated_nominal_unit=W  fidelity_level=ee.enum.diode.fidelity.includeChargeDyn  rec_loss_model=ee.enum.diode.reverseRecoveryModel.fixed  ErecVal=0 J  scaleWithIandV=true  ErecMat=zeros(2, 3) J  TjrecVec=[298.15, 398.15] K  IfrecVec=[.1, 1, 10] A  IrecVal=10 A  VrecVal=10 V  tFilter=1 / 1000 / 100 s  thermal_network_parameterization=ee.enum.thermalNetworkTopology.junctionCase  Rth=[0, 10] K/W  Rth_Cauer=[1, 3, 10] K/W  Rth_Foster=[.08, .14, .22, .16] K/W  thermal_mass_parameterization=ee.enum.thermalNetwork.timeconstant  thermal_mass=[0, 1] J/K  thermal_mass_Cauer=[.1, .3, 1] J/K  thermal_mass_Foster=[.001, .005, .05, .5] J/K  thermal_time_constant=[0, 10] s  thermal_time_constant_Cauer=[1, 3, 10] s  thermal_time_constant_Foster=[7e-05, .0007, .01, .08] s  thermal_mass_initial_temperatures=[25, 25] degC  thermal_mass_initial_temperatures_Cauer=[25, 25, 25] degC  junction_thermal_mass=0.01 J/K  Tvec_initial_Foster=[25, 25, 25, 25] degC  no_thermal_network=0  junction_temperature_specify=off  junction_temperature_priority=None  junction_temperature=25 degC  junction_temperature_nominal_specify=off  junction_temperature_nominal_value=1  junction_temperature_nominal_unit=degC
  D_44_3 : ee_lib/Semiconductors & Converters/Diode  ModelType=ee.enum.diode.modelType.pwl  TableType=ee.enum.diode.tableType.IfMat  IfMat=[.07, .12, .19, 1.75, 4.24, 7.32, 11.2; .16, .3, .72, 2.14, 5.02, 8.35, 13.12] A  VfMat=[.9, 1.15, 1.25, 1.5, 1.75, 2.17, 2.6, 2.85; .58, .68, .75, 1.1, 1.38, 1.77, 2.27, 2.7] V  TjVec=[25, 125] degC  VfVec=[.5, .7, .9, 1.3, 1.7, 2.1, 2.5] V  IfVec=[.1, .2, .5, 1, 2, 4, 7, 10] A  IrMat=[1e-06, 2e-06, 5e-06, 1e-05, 2.5e-05, 5e-05, .0001; 2e-06, 5e-06, 1e-05, 4e-05, 8e-05, .0002, .0005] A  VrMat=[10, 100, 200, 250, 300, 325, 350; 10, 70, 160, 220, 270, 300, 320] V  VrVec=[10, 20, 40, 50, 70, 80, 100] V  IrVec=[1e-06, 2e-06, 5e-06, 1e-05, 2e-05, 5e-05, .0001] A  Vf=byp_Vf V  Ron=byp_Ron Ohm  Goff=byp_Goff S  prmExp=ee.enum.diode.expParam.useTwo  I12=[.0137, .545] A  V12=[.6, .7] V  RS=0 Ohm  Tmeas=298.15 K  IS=1e-12 A  ec=1  I1=0.0137 A  V1=0.6 V  N_series=1  N_parallel=1  ZenerEnable=false  Rz=0.3 Ohm  BV=inf V  C_param=ee.enum.diode.capParam.fixed  CJ=0 pF  CJ0=5 pF  Vvec=[.1, 10, 100] V  Cvec=[3.5, 1, .4] pF  VJ=1 V  Mgrad=0.5  FC=0.5  Q_param=ee.enum.diode.recoveryParam.off  iRM=-7.15 A  iF=4 A  didt=-750 A/us  trr_factor=3  trr=115 ns  Qrr=150 nA*s  Vr=-600 V  Ls=150 nH  Erec=0.03 J  TT=50 ns  tau=100 ns  T_param=ee.enum.diode.temperatureParam.off  Tdevice=298.15 K  I1_T2=0.245 A  V1_T2=0.5 V  IS_T2=1.25e-7 A  Tmeas2=125 degC  XTI_param=ee.enum.diode.xtiParam.pn  XTI=3  EG_param=ee.enum.diode.egapParam.material_si  EG=1.11 eV  dBVdT=0 V/K  enable_fault_input=simscape.enum.onoff.off  i_specify=off  i_priority=None  i=0 A  i_nominal_specify=off  i_nominal_value=1  i_nominal_unit=A  v_specify=off  v_priority=None  v=0 V  v_nominal_specify=off  v_nominal_value=1  v_nominal_unit=V  v_capacitor_specify=off  v_capacitor_priority=None  v_capacitor=0 V  v_capacitor_nominal_specify=off  v_capacitor_nominal_value=1  v_capacitor_nominal_unit=V  Qj_specify=off  Qj_priority=High  Qj=0 C  Qj_nominal_specify=off  Qj_nominal_value=1  Qj_nominal_unit=C  i_diode_specify=off  i_diode_priority=None  i_diode=0 A  i_diode_nominal_specify=off  i_diode_nominal_value=1  i_diode_nominal_unit=A  v_diode_specify=off  v_diode_priority=None  v_diode=0 V  v_diode_nominal_specify=off  v_diode_nominal_value=1  v_diode_nominal_unit=V  i_capacitor_specify=off  i_capacitor_priority=None  i_capacitor=0 A  i_capacitor_nominal_specify=off  i_capacitor_nominal_value=1  i_capacitor_nominal_unit=A  power_dissipated_specify=off  power_dissipated_priority=None  power_dissipated=0 W  power_dissipated_nominal_specify=off  power_dissipated_nominal_value=1  power_dissipated_nominal_unit=W  fidelity_level=ee.enum.diode.fidelity.includeChargeDyn  rec_loss_model=ee.enum.diode.reverseRecoveryModel.fixed  ErecVal=0 J  scaleWithIandV=true  ErecMat=zeros(2, 3) J  TjrecVec=[298.15, 398.15] K  IfrecVec=[.1, 1, 10] A  IrecVal=10 A  VrecVal=10 V  tFilter=1 / 1000 / 100 s  thermal_network_parameterization=ee.enum.thermalNetworkTopology.junctionCase  Rth=[0, 10] K/W  Rth_Cauer=[1, 3, 10] K/W  Rth_Foster=[.08, .14, .22, .16] K/W  thermal_mass_parameterization=ee.enum.thermalNetwork.timeconstant  thermal_mass=[0, 1] J/K  thermal_mass_Cauer=[.1, .3, 1] J/K  thermal_mass_Foster=[.001, .005, .05, .5] J/K  thermal_time_constant=[0, 10] s  thermal_time_constant_Cauer=[1, 3, 10] s  thermal_time_constant_Foster=[7e-05, .0007, .01, .08] s  thermal_mass_initial_temperatures=[25, 25] degC  thermal_mass_initial_temperatures_Cauer=[25, 25, 25] degC  junction_thermal_mass=0.01 J/K  Tvec_initial_Foster=[25, 25, 25, 25] degC  no_thermal_network=0  junction_temperature_specify=off  junction_temperature_priority=None  junction_temperature=25 degC  junction_temperature_nominal_specify=off  junction_temperature_nominal_value=1  junction_temperature_nominal_unit=degC
  Demux : Demux  Outputs=48
  G_11_1 : nesl_utility/Simulink-PS Converter  PhysicalDomain=network_engine_domain  SubClassName=ps_input  LeftPortType=input  RightPortType=output  PseudoPeriodic=off  Frequencies=[]  NoiseDistribution=none  NoiseParameters=[]  Unit=W/m^2  AffineConversion=off  FilteringAndDerivatives=filter  SimscapeFilterOrder=1  InputFilterTimeConstant=G_tau  UdotUserProvided=0
  G_11_2 : nesl_utility/Simulink-PS Converter  PhysicalDomain=network_engine_domain  SubClassName=ps_input  LeftPortType=input  RightPortType=output  PseudoPeriodic=off  Frequencies=[]  NoiseDistribution=none  NoiseParameters=[]  Unit=W/m^2  AffineConversion=off  FilteringAndDerivatives=filter  SimscapeFilterOrder=1  InputFilterTimeConstant=G_tau  UdotUserProvided=0
  G_11_3 : nesl_utility/Simulink-PS Converter  PhysicalDomain=network_engine_domain  SubClassName=ps_input  LeftPortType=input  RightPortType=output  PseudoPeriodic=off  Frequencies=[]  NoiseDistribution=none  NoiseParameters=[]  Unit=W/m^2  AffineConversion=off  FilteringAndDerivatives=filter  SimscapeFilterOrder=1  InputFilterTimeConstant=G_tau  UdotUserProvided=0
  G_12_1 : nesl_utility/Simulink-PS Converter  PhysicalDomain=network_engine_domain  SubClassName=ps_input  LeftPortType=input  RightPortType=output  PseudoPeriodic=off  Frequencies=[]  NoiseDistribution=none  NoiseParameters=[]  Unit=W/m^2  AffineConversion=off  FilteringAndDerivatives=filter  SimscapeFilterOrder=1  InputFilterTimeConstant=G_tau  UdotUserProvided=0
  G_12_2 : nesl_utility/Simulink-PS Converter  PhysicalDomain=network_engine_domain  SubClassName=ps_input  LeftPortType=input  RightPortType=output  PseudoPeriodic=off  Frequencies=[]  NoiseDistribution=none  NoiseParameters=[]  Unit=W/m^2  AffineConversion=off  FilteringAndDerivatives=filter  SimscapeFilterOrder=1  InputFilterTimeConstant=G_tau  UdotUserProvided=0
  G_12_3 : nesl_utility/Simulink-PS Converter  PhysicalDomain=network_engine_domain  SubClassName=ps_input  LeftPortType=input  RightPortType=output  PseudoPeriodic=off  Frequencies=[]  NoiseDistribution=none  NoiseParameters=[]  Unit=W/m^2  AffineConversion=off  FilteringAndDerivatives=filter  SimscapeFilterOrder=1  InputFilterTimeConstant=G_tau  UdotUserProvided=0
  G_13_1 : nesl_utility/Simulink-PS Converter  PhysicalDomain=network_engine_domain  SubClassName=ps_input  LeftPortType=input  RightPortType=output  PseudoPeriodic=off  Frequencies=[]  NoiseDistribution=none  NoiseParameters=[]  Unit=W/m^2  AffineConversion=off  FilteringAndDerivatives=filter  SimscapeFilterOrder=1  InputFilterTimeConstant=G_tau  UdotUserProvided=0
  G_13_2 : nesl_utility/Simulink-PS Converter  PhysicalDomain=network_engine_domain  SubClassName=ps_input  LeftPortType=input  RightPortType=output  PseudoPeriodic=off  Frequencies=[]  NoiseDistribution=none  NoiseParameters=[]  Unit=W/m^2  AffineConversion=off  FilteringAndDerivatives=filter  SimscapeFilterOrder=1  InputFilterTimeConstant=G_tau  UdotUserProvided=0
  G_13_3 : nesl_utility/Simulink-PS Converter  PhysicalDomain=network_engine_domain  SubClassName=ps_input  LeftPortType=input  RightPortType=output  PseudoPeriodic=off  Frequencies=[]  NoiseDistribution=none  NoiseParameters=[]  Unit=W/m^2  AffineConversion=off  FilteringAndDerivatives=filter  SimscapeFilterOrder=1  InputFilterTimeConstant=G_tau  UdotUserProvided=0
  G_14_1 : nesl_utility/Simulink-PS Converter  PhysicalDomain=network_engine_domain  SubClassName=ps_input  LeftPortType=input  RightPortType=output  PseudoPeriodic=off  Frequencies=[]  NoiseDistribution=none  NoiseParameters=[]  Unit=W/m^2  AffineConversion=off  FilteringAndDerivatives=filter  SimscapeFilterOrder=1  InputFilterTimeConstant=G_tau  UdotUserProvided=0
  G_14_2 : nesl_utility/Simulink-PS Converter  PhysicalDomain=network_engine_domain  SubClassName=ps_input  LeftPortType=input  RightPortType=output  PseudoPeriodic=off  Frequencies=[]  NoiseDistribution=none  NoiseParameters=[]  Unit=W/m^2  AffineConversion=off  FilteringAndDerivatives=filter  SimscapeFilterOrder=1  InputFilterTimeConstant=G_tau  UdotUserProvided=0
  G_14_3 : nesl_utility/Simulink-PS Converter  PhysicalDomain=network_engine_domain  SubClassName=ps_input  LeftPortType=input  RightPortType=output  PseudoPeriodic=off  Frequencies=[]  NoiseDistribution=none  NoiseParameters=[]  Unit=W/m^2  AffineConversion=off  FilteringAndDerivatives=filter  SimscapeFilterOrder=1  InputFilterTimeConstant=G_tau  UdotUserProvided=0
  G_21_1 : nesl_utility/Simulink-PS Converter  PhysicalDomain=network_engine_domain  SubClassName=ps_input  LeftPortType=input  RightPortType=output  PseudoPeriodic=off  Frequencies=[]  NoiseDistribution=none  NoiseParameters=[]  Unit=W/m^2  AffineConversion=off  FilteringAndDerivatives=filter  SimscapeFilterOrder=1  InputFilterTimeConstant=G_tau  UdotUserProvided=0
  G_21_2 : nesl_utility/Simulink-PS Converter  PhysicalDomain=network_engine_domain  SubClassName=ps_input  LeftPortType=input  RightPortType=output  PseudoPeriodic=off  Frequencies=[]  NoiseDistribution=none  NoiseParameters=[]  Unit=W/m^2  AffineConversion=off  FilteringAndDerivatives=filter  SimscapeFilterOrder=1  InputFilterTimeConstant=G_tau  UdotUserProvided=0
  G_21_3 : nesl_utility/Simulink-PS Converter  PhysicalDomain=network_engine_domain  SubClassName=ps_input  LeftPortType=input  RightPortType=output  PseudoPeriodic=off  Frequencies=[]  NoiseDistribution=none  NoiseParameters=[]  Unit=W/m^2  AffineConversion=off  FilteringAndDerivatives=filter  SimscapeFilterOrder=1  InputFilterTimeConstant=G_tau  UdotUserProvided=0
  G_22_1 : nesl_utility/Simulink-PS Converter  PhysicalDomain=network_engine_domain  SubClassName=ps_input  LeftPortType=input  RightPortType=output  PseudoPeriodic=off  Frequencies=[]  NoiseDistribution=none  NoiseParameters=[]  Unit=W/m^2  AffineConversion=off  FilteringAndDerivatives=filter  SimscapeFilterOrder=1  InputFilterTimeConstant=G_tau  UdotUserProvided=0
  G_22_2 : nesl_utility/Simulink-PS Converter  PhysicalDomain=network_engine_domain  SubClassName=ps_input  LeftPortType=input  RightPortType=output  PseudoPeriodic=off  Frequencies=[]  NoiseDistribution=none  NoiseParameters=[]  Unit=W/m^2  AffineConversion=off  FilteringAndDerivatives=filter  SimscapeFilterOrder=1  InputFilterTimeConstant=G_tau  UdotUserProvided=0
  G_22_3 : nesl_utility/Simulink-PS Converter  PhysicalDomain=network_engine_domain  SubClassName=ps_input  LeftPortType=input  RightPortType=output  PseudoPeriodic=off  Frequencies=[]  NoiseDistribution=none  NoiseParameters=[]  Unit=W/m^2  AffineConversion=off  FilteringAndDerivatives=filter  SimscapeFilterOrder=1  InputFilterTimeConstant=G_tau  UdotUserProvided=0
  G_23_1 : nesl_utility/Simulink-PS Converter  PhysicalDomain=network_engine_domain  SubClassName=ps_input  LeftPortType=input  RightPortType=output  PseudoPeriodic=off  Frequencies=[]  NoiseDistribution=none  NoiseParameters=[]  Unit=W/m^2  AffineConversion=off  FilteringAndDerivatives=filter  SimscapeFilterOrder=1  InputFilterTimeConstant=G_tau  UdotUserProvided=0
  G_23_2 : nesl_utility/Simulink-PS Converter  PhysicalDomain=network_engine_domain  SubClassName=ps_input  LeftPortType=input  RightPortType=output  PseudoPeriodic=off  Frequencies=[]  NoiseDistribution=none  NoiseParameters=[]  Unit=W/m^2  AffineConversion=off  FilteringAndDerivatives=filter  SimscapeFilterOrder=1  InputFilterTimeConstant=G_tau  UdotUserProvided=0
  G_23_3 : nesl_utility/Simulink-PS Converter  PhysicalDomain=network_engine_domain  SubClassName=ps_input  LeftPortType=input  RightPortType=output  PseudoPeriodic=off  Frequencies=[]  NoiseDistribution=none  NoiseParameters=[]  Unit=W/m^2  AffineConversion=off  FilteringAndDerivatives=filter  SimscapeFilterOrder=1  InputFilterTimeConstant=G_tau  UdotUserProvided=0
  G_24_1 : nesl_utility/Simulink-PS Converter  PhysicalDomain=network_engine_domain  SubClassName=ps_input  LeftPortType=input  RightPortType=output  PseudoPeriodic=off  Frequencies=[]  NoiseDistribution=none  NoiseParameters=[]  Unit=W/m^2  AffineConversion=off  FilteringAndDerivatives=filter  SimscapeFilterOrder=1  InputFilterTimeConstant=G_tau  UdotUserProvided=0
  G_24_2 : nesl_utility/Simulink-PS Converter  PhysicalDomain=network_engine_domain  SubClassName=ps_input  LeftPortType=input  RightPortType=output  PseudoPeriodic=off  Frequencies=[]  NoiseDistribution=none  NoiseParameters=[]  Unit=W/m^2  AffineConversion=off  FilteringAndDerivatives=filter  SimscapeFilterOrder=1  InputFilterTimeConstant=G_tau  UdotUserProvided=0
  G_24_3 : nesl_utility/Simulink-PS Converter  PhysicalDomain=network_engine_domain  SubClassName=ps_input  LeftPortType=input  RightPortType=output  PseudoPeriodic=off  Frequencies=[]  NoiseDistribution=none  NoiseParameters=[]  Unit=W/m^2  AffineConversion=off  FilteringAndDerivatives=filter  SimscapeFilterOrder=1  InputFilterTimeConstant=G_tau  UdotUserProvided=0
  G_31_1 : nesl_utility/Simulink-PS Converter  PhysicalDomain=network_engine_domain  SubClassName=ps_input  LeftPortType=input  RightPortType=output  PseudoPeriodic=off  Frequencies=[]  NoiseDistribution=none  NoiseParameters=[]  Unit=W/m^2  AffineConversion=off  FilteringAndDerivatives=filter  SimscapeFilterOrder=1  InputFilterTimeConstant=G_tau  UdotUserProvided=0
  G_31_2 : nesl_utility/Simulink-PS Converter  PhysicalDomain=network_engine_domain  SubClassName=ps_input  LeftPortType=input  RightPortType=output  PseudoPeriodic=off  Frequencies=[]  NoiseDistribution=none  NoiseParameters=[]  Unit=W/m^2  AffineConversion=off  FilteringAndDerivatives=filter  SimscapeFilterOrder=1  InputFilterTimeConstant=G_tau  UdotUserProvided=0
  G_31_3 : nesl_utility/Simulink-PS Converter  PhysicalDomain=network_engine_domain  SubClassName=ps_input  LeftPortType=input  RightPortType=output  PseudoPeriodic=off  Frequencies=[]  NoiseDistribution=none  NoiseParameters=[]  Unit=W/m^2  AffineConversion=off  FilteringAndDerivatives=filter  SimscapeFilterOrder=1  InputFilterTimeConstant=G_tau  UdotUserProvided=0
  G_32_1 : nesl_utility/Simulink-PS Converter  PhysicalDomain=network_engine_domain  SubClassName=ps_input  LeftPortType=input  RightPortType=output  PseudoPeriodic=off  Frequencies=[]  NoiseDistribution=none  NoiseParameters=[]  Unit=W/m^2  AffineConversion=off  FilteringAndDerivatives=filter  SimscapeFilterOrder=1  InputFilterTimeConstant=G_tau  UdotUserProvided=0
  G_32_2 : nesl_utility/Simulink-PS Converter  PhysicalDomain=network_engine_domain  SubClassName=ps_input  LeftPortType=input  RightPortType=output  PseudoPeriodic=off  Frequencies=[]  NoiseDistribution=none  NoiseParameters=[]  Unit=W/m^2  AffineConversion=off  FilteringAndDerivatives=filter  SimscapeFilterOrder=1  InputFilterTimeConstant=G_tau  UdotUserProvided=0
  G_32_3 : nesl_utility/Simulink-PS Converter  PhysicalDomain=network_engine_domain  SubClassName=ps_input  LeftPortType=input  RightPortType=output  PseudoPeriodic=off  Frequencies=[]  NoiseDistribution=none  NoiseParameters=[]  Unit=W/m^2  AffineConversion=off  FilteringAndDerivatives=filter  SimscapeFilterOrder=1  InputFilterTimeConstant=G_tau  UdotUserProvided=0
  G_33_1 : nesl_utility/Simulink-PS Converter  PhysicalDomain=network_engine_domain  SubClassName=ps_input  LeftPortType=input  RightPortType=output  PseudoPeriodic=off  Frequencies=[]  NoiseDistribution=none  NoiseParameters=[]  Unit=W/m^2  AffineConversion=off  FilteringAndDerivatives=filter  SimscapeFilterOrder=1  InputFilterTimeConstant=G_tau  UdotUserProvided=0
  G_33_2 : nesl_utility/Simulink-PS Converter  PhysicalDomain=network_engine_domain  SubClassName=ps_input  LeftPortType=input  RightPortType=output  PseudoPeriodic=off  Frequencies=[]  NoiseDistribution=none  NoiseParameters=[]  Unit=W/m^2  AffineConversion=off  FilteringAndDerivatives=filter  SimscapeFilterOrder=1  InputFilterTimeConstant=G_tau  UdotUserProvided=0
  G_33_3 : nesl_utility/Simulink-PS Converter  PhysicalDomain=network_engine_domain  SubClassName=ps_input  LeftPortType=input  RightPortType=output  PseudoPeriodic=off  Frequencies=[]  NoiseDistribution=none  NoiseParameters=[]  Unit=W/m^2  AffineConversion=off  FilteringAndDerivatives=filter  SimscapeFilterOrder=1  InputFilterTimeConstant=G_tau  UdotUserProvided=0
  G_34_1 : nesl_utility/Simulink-PS Converter  PhysicalDomain=network_engine_domain  SubClassName=ps_input  LeftPortType=input  RightPortType=output  PseudoPeriodic=off  Frequencies=[]  NoiseDistribution=none  NoiseParameters=[]  Unit=W/m^2  AffineConversion=off  FilteringAndDerivatives=filter  SimscapeFilterOrder=1  InputFilterTimeConstant=G_tau  UdotUserProvided=0
  G_34_2 : nesl_utility/Simulink-PS Converter  PhysicalDomain=network_engine_domain  SubClassName=ps_input  LeftPortType=input  RightPortType=output  PseudoPeriodic=off  Frequencies=[]  NoiseDistribution=none  NoiseParameters=[]  Unit=W/m^2  AffineConversion=off  FilteringAndDerivatives=filter  SimscapeFilterOrder=1  InputFilterTimeConstant=G_tau  UdotUserProvided=0
  G_34_3 : nesl_utility/Simulink-PS Converter  PhysicalDomain=network_engine_domain  SubClassName=ps_input  LeftPortType=input  RightPortType=output  PseudoPeriodic=off  Frequencies=[]  NoiseDistribution=none  NoiseParameters=[]  Unit=W/m^2  AffineConversion=off  FilteringAndDerivatives=filter  SimscapeFilterOrder=1  InputFilterTimeConstant=G_tau  UdotUserProvided=0
  G_41_1 : nesl_utility/Simulink-PS Converter  PhysicalDomain=network_engine_domain  SubClassName=ps_input  LeftPortType=input  RightPortType=output  PseudoPeriodic=off  Frequencies=[]  NoiseDistribution=none  NoiseParameters=[]  Unit=W/m^2  AffineConversion=off  FilteringAndDerivatives=filter  SimscapeFilterOrder=1  InputFilterTimeConstant=G_tau  UdotUserProvided=0
  G_41_2 : nesl_utility/Simulink-PS Converter  PhysicalDomain=network_engine_domain  SubClassName=ps_input  LeftPortType=input  RightPortType=output  PseudoPeriodic=off  Frequencies=[]  NoiseDistribution=none  NoiseParameters=[]  Unit=W/m^2  AffineConversion=off  FilteringAndDerivatives=filter  SimscapeFilterOrder=1  InputFilterTimeConstant=G_tau  UdotUserProvided=0
  G_41_3 : nesl_utility/Simulink-PS Converter  PhysicalDomain=network_engine_domain  SubClassName=ps_input  LeftPortType=input  RightPortType=output  PseudoPeriodic=off  Frequencies=[]  NoiseDistribution=none  NoiseParameters=[]  Unit=W/m^2  AffineConversion=off  FilteringAndDerivatives=filter  SimscapeFilterOrder=1  InputFilterTimeConstant=G_tau  UdotUserProvided=0
  G_42_1 : nesl_utility/Simulink-PS Converter  PhysicalDomain=network_engine_domain  SubClassName=ps_input  LeftPortType=input  RightPortType=output  PseudoPeriodic=off  Frequencies=[]  NoiseDistribution=none  NoiseParameters=[]  Unit=W/m^2  AffineConversion=off  FilteringAndDerivatives=filter  SimscapeFilterOrder=1  InputFilterTimeConstant=G_tau  UdotUserProvided=0
  G_42_2 : nesl_utility/Simulink-PS Converter  PhysicalDomain=network_engine_domain  SubClassName=ps_input  LeftPortType=input  RightPortType=output  PseudoPeriodic=off  Frequencies=[]  NoiseDistribution=none  NoiseParameters=[]  Unit=W/m^2  AffineConversion=off  FilteringAndDerivatives=filter  SimscapeFilterOrder=1  InputFilterTimeConstant=G_tau  UdotUserProvided=0
  G_42_3 : nesl_utility/Simulink-PS Converter  PhysicalDomain=network_engine_domain  SubClassName=ps_input  LeftPortType=input  RightPortType=output  PseudoPeriodic=off  Frequencies=[]  NoiseDistribution=none  NoiseParameters=[]  Unit=W/m^2  AffineConversion=off  FilteringAndDerivatives=filter  SimscapeFilterOrder=1  InputFilterTimeConstant=G_tau  UdotUserProvided=0
  G_43_1 : nesl_utility/Simulink-PS Converter  PhysicalDomain=network_engine_domain  SubClassName=ps_input  LeftPortType=input  RightPortType=output  PseudoPeriodic=off  Frequencies=[]  NoiseDistribution=none  NoiseParameters=[]  Unit=W/m^2  AffineConversion=off  FilteringAndDerivatives=filter  SimscapeFilterOrder=1  InputFilterTimeConstant=G_tau  UdotUserProvided=0
  G_43_2 : nesl_utility/Simulink-PS Converter  PhysicalDomain=network_engine_domain  SubClassName=ps_input  LeftPortType=input  RightPortType=output  PseudoPeriodic=off  Frequencies=[]  NoiseDistribution=none  NoiseParameters=[]  Unit=W/m^2  AffineConversion=off  FilteringAndDerivatives=filter  SimscapeFilterOrder=1  InputFilterTimeConstant=G_tau  UdotUserProvided=0
  G_43_3 : nesl_utility/Simulink-PS Converter  PhysicalDomain=network_engine_domain  SubClassName=ps_input  LeftPortType=input  RightPortType=output  PseudoPeriodic=off  Frequencies=[]  NoiseDistribution=none  NoiseParameters=[]  Unit=W/m^2  AffineConversion=off  FilteringAndDerivatives=filter  SimscapeFilterOrder=1  InputFilterTimeConstant=G_tau  UdotUserProvided=0
  G_44_1 : nesl_utility/Simulink-PS Converter  PhysicalDomain=network_engine_domain  SubClassName=ps_input  LeftPortType=input  RightPortType=output  PseudoPeriodic=off  Frequencies=[]  NoiseDistribution=none  NoiseParameters=[]  Unit=W/m^2  AffineConversion=off  FilteringAndDerivatives=filter  SimscapeFilterOrder=1  InputFilterTimeConstant=G_tau  UdotUserProvided=0
  G_44_2 : nesl_utility/Simulink-PS Converter  PhysicalDomain=network_engine_domain  SubClassName=ps_input  LeftPortType=input  RightPortType=output  PseudoPeriodic=off  Frequencies=[]  NoiseDistribution=none  NoiseParameters=[]  Unit=W/m^2  AffineConversion=off  FilteringAndDerivatives=filter  SimscapeFilterOrder=1  InputFilterTimeConstant=G_tau  UdotUserProvided=0
  G_44_3 : nesl_utility/Simulink-PS Converter  PhysicalDomain=network_engine_domain  SubClassName=ps_input  LeftPortType=input  RightPortType=output  PseudoPeriodic=off  Frequencies=[]  NoiseDistribution=none  NoiseParameters=[]  Unit=W/m^2  AffineConversion=off  FilteringAndDerivatives=filter  SimscapeFilterOrder=1  InputFilterTimeConstant=G_tau  UdotUserProvided=0
  PV_11_1 : ee_lib/Sources/Solar Cell  prm=ee.enum.sources.solar_cell_prm.datasheet  Isc=pv_Isc A  Voc=pv_Voc V  Is=1e-6 A  Is2=0 A  Iph=7.34 A  Ir0=pv_Ir0 W/m^2  ec=pv_n  N2=2  Rs=pv_Rs Ohm  Rp=inf Ohm  N_series=pv_Ngrp  N_parallel=1  TIPH1=pv_TIPH1 1/K  EG=pv_EG eV  TXIS1=pv_TXIS1  TXIS2=3  TRS1=pv_TRS1  TRP1=0  Tmeas=pv_Tmeas degC  TFIXED=pv_T degC  thermal_mass=100 J/K  initial_temperature=25 degC
  PV_11_2 : ee_lib/Sources/Solar Cell  prm=ee.enum.sources.solar_cell_prm.datasheet  Isc=pv_Isc A  Voc=pv_Voc V  Is=1e-6 A  Is2=0 A  Iph=7.34 A  Ir0=pv_Ir0 W/m^2  ec=pv_n  N2=2  Rs=pv_Rs Ohm  Rp=inf Ohm  N_series=pv_Ngrp  N_parallel=1  TIPH1=pv_TIPH1 1/K  EG=pv_EG eV  TXIS1=pv_TXIS1  TXIS2=3  TRS1=pv_TRS1  TRP1=0  Tmeas=pv_Tmeas degC  TFIXED=pv_T degC  thermal_mass=100 J/K  initial_temperature=25 degC
  PV_11_3 : ee_lib/Sources/Solar Cell  prm=ee.enum.sources.solar_cell_prm.datasheet  Isc=pv_Isc A  Voc=pv_Voc V  Is=1e-6 A  Is2=0 A  Iph=7.34 A  Ir0=pv_Ir0 W/m^2  ec=pv_n  N2=2  Rs=pv_Rs Ohm  Rp=inf Ohm  N_series=pv_Ngrp  N_parallel=1  TIPH1=pv_TIPH1 1/K  EG=pv_EG eV  TXIS1=pv_TXIS1  TXIS2=3  TRS1=pv_TRS1  TRP1=0  Tmeas=pv_Tmeas degC  TFIXED=pv_T degC  thermal_mass=100 J/K  initial_temperature=25 degC
  PV_12_1 : ee_lib/Sources/Solar Cell  prm=ee.enum.sources.solar_cell_prm.datasheet  Isc=pv_Isc A  Voc=pv_Voc V  Is=1e-6 A  Is2=0 A  Iph=7.34 A  Ir0=pv_Ir0 W/m^2  ec=pv_n  N2=2  Rs=pv_Rs Ohm  Rp=inf Ohm  N_series=pv_Ngrp  N_parallel=1  TIPH1=pv_TIPH1 1/K  EG=pv_EG eV  TXIS1=pv_TXIS1  TXIS2=3  TRS1=pv_TRS1  TRP1=0  Tmeas=pv_Tmeas degC  TFIXED=pv_T degC  thermal_mass=100 J/K  initial_temperature=25 degC
  PV_12_2 : ee_lib/Sources/Solar Cell  prm=ee.enum.sources.solar_cell_prm.datasheet  Isc=pv_Isc A  Voc=pv_Voc V  Is=1e-6 A  Is2=0 A  Iph=7.34 A  Ir0=pv_Ir0 W/m^2  ec=pv_n  N2=2  Rs=pv_Rs Ohm  Rp=inf Ohm  N_series=pv_Ngrp  N_parallel=1  TIPH1=pv_TIPH1 1/K  EG=pv_EG eV  TXIS1=pv_TXIS1  TXIS2=3  TRS1=pv_TRS1  TRP1=0  Tmeas=pv_Tmeas degC  TFIXED=pv_T degC  thermal_mass=100 J/K  initial_temperature=25 degC
  PV_12_3 : ee_lib/Sources/Solar Cell  prm=ee.enum.sources.solar_cell_prm.datasheet  Isc=pv_Isc A  Voc=pv_Voc V  Is=1e-6 A  Is2=0 A  Iph=7.34 A  Ir0=pv_Ir0 W/m^2  ec=pv_n  N2=2  Rs=pv_Rs Ohm  Rp=inf Ohm  N_series=pv_Ngrp  N_parallel=1  TIPH1=pv_TIPH1 1/K  EG=pv_EG eV  TXIS1=pv_TXIS1  TXIS2=3  TRS1=pv_TRS1  TRP1=0  Tmeas=pv_Tmeas degC  TFIXED=pv_T degC  thermal_mass=100 J/K  initial_temperature=25 degC
  PV_13_1 : ee_lib/Sources/Solar Cell  prm=ee.enum.sources.solar_cell_prm.datasheet  Isc=pv_Isc A  Voc=pv_Voc V  Is=1e-6 A  Is2=0 A  Iph=7.34 A  Ir0=pv_Ir0 W/m^2  ec=pv_n  N2=2  Rs=pv_Rs Ohm  Rp=inf Ohm  N_series=pv_Ngrp  N_parallel=1  TIPH1=pv_TIPH1 1/K  EG=pv_EG eV  TXIS1=pv_TXIS1  TXIS2=3  TRS1=pv_TRS1  TRP1=0  Tmeas=pv_Tmeas degC  TFIXED=pv_T degC  thermal_mass=100 J/K  initial_temperature=25 degC
  PV_13_2 : ee_lib/Sources/Solar Cell  prm=ee.enum.sources.solar_cell_prm.datasheet  Isc=pv_Isc A  Voc=pv_Voc V  Is=1e-6 A  Is2=0 A  Iph=7.34 A  Ir0=pv_Ir0 W/m^2  ec=pv_n  N2=2  Rs=pv_Rs Ohm  Rp=inf Ohm  N_series=pv_Ngrp  N_parallel=1  TIPH1=pv_TIPH1 1/K  EG=pv_EG eV  TXIS1=pv_TXIS1  TXIS2=3  TRS1=pv_TRS1  TRP1=0  Tmeas=pv_Tmeas degC  TFIXED=pv_T degC  thermal_mass=100 J/K  initial_temperature=25 degC
  PV_13_3 : ee_lib/Sources/Solar Cell  prm=ee.enum.sources.solar_cell_prm.datasheet  Isc=pv_Isc A  Voc=pv_Voc V  Is=1e-6 A  Is2=0 A  Iph=7.34 A  Ir0=pv_Ir0 W/m^2  ec=pv_n  N2=2  Rs=pv_Rs Ohm  Rp=inf Ohm  N_series=pv_Ngrp  N_parallel=1  TIPH1=pv_TIPH1 1/K  EG=pv_EG eV  TXIS1=pv_TXIS1  TXIS2=3  TRS1=pv_TRS1  TRP1=0  Tmeas=pv_Tmeas degC  TFIXED=pv_T degC  thermal_mass=100 J/K  initial_temperature=25 degC
  PV_14_1 : ee_lib/Sources/Solar Cell  prm=ee.enum.sources.solar_cell_prm.datasheet  Isc=pv_Isc A  Voc=pv_Voc V  Is=1e-6 A  Is2=0 A  Iph=7.34 A  Ir0=pv_Ir0 W/m^2  ec=pv_n  N2=2  Rs=pv_Rs Ohm  Rp=inf Ohm  N_series=pv_Ngrp  N_parallel=1  TIPH1=pv_TIPH1 1/K  EG=pv_EG eV  TXIS1=pv_TXIS1  TXIS2=3  TRS1=pv_TRS1  TRP1=0  Tmeas=pv_Tmeas degC  TFIXED=pv_T degC  thermal_mass=100 J/K  initial_temperature=25 degC
  PV_14_2 : ee_lib/Sources/Solar Cell  prm=ee.enum.sources.solar_cell_prm.datasheet  Isc=pv_Isc A  Voc=pv_Voc V  Is=1e-6 A  Is2=0 A  Iph=7.34 A  Ir0=pv_Ir0 W/m^2  ec=pv_n  N2=2  Rs=pv_Rs Ohm  Rp=inf Ohm  N_series=pv_Ngrp  N_parallel=1  TIPH1=pv_TIPH1 1/K  EG=pv_EG eV  TXIS1=pv_TXIS1  TXIS2=3  TRS1=pv_TRS1  TRP1=0  Tmeas=pv_Tmeas degC  TFIXED=pv_T degC  thermal_mass=100 J/K  initial_temperature=25 degC
  PV_14_3 : ee_lib/Sources/Solar Cell  prm=ee.enum.sources.solar_cell_prm.datasheet  Isc=pv_Isc A  Voc=pv_Voc V  Is=1e-6 A  Is2=0 A  Iph=7.34 A  Ir0=pv_Ir0 W/m^2  ec=pv_n  N2=2  Rs=pv_Rs Ohm  Rp=inf Ohm  N_series=pv_Ngrp  N_parallel=1  TIPH1=pv_TIPH1 1/K  EG=pv_EG eV  TXIS1=pv_TXIS1  TXIS2=3  TRS1=pv_TRS1  TRP1=0  Tmeas=pv_Tmeas degC  TFIXED=pv_T degC  thermal_mass=100 J/K  initial_temperature=25 degC
  PV_21_1 : ee_lib/Sources/Solar Cell  prm=ee.enum.sources.solar_cell_prm.datasheet  Isc=pv_Isc A  Voc=pv_Voc V  Is=1e-6 A  Is2=0 A  Iph=7.34 A  Ir0=pv_Ir0 W/m^2  ec=pv_n  N2=2  Rs=pv_Rs Ohm  Rp=inf Ohm  N_series=pv_Ngrp  N_parallel=1  TIPH1=pv_TIPH1 1/K  EG=pv_EG eV  TXIS1=pv_TXIS1  TXIS2=3  TRS1=pv_TRS1  TRP1=0  Tmeas=pv_Tmeas degC  TFIXED=pv_T degC  thermal_mass=100 J/K  initial_temperature=25 degC
  PV_21_2 : ee_lib/Sources/Solar Cell  prm=ee.enum.sources.solar_cell_prm.datasheet  Isc=pv_Isc A  Voc=pv_Voc V  Is=1e-6 A  Is2=0 A  Iph=7.34 A  Ir0=pv_Ir0 W/m^2  ec=pv_n  N2=2  Rs=pv_Rs Ohm  Rp=inf Ohm  N_series=pv_Ngrp  N_parallel=1  TIPH1=pv_TIPH1 1/K  EG=pv_EG eV  TXIS1=pv_TXIS1  TXIS2=3  TRS1=pv_TRS1  TRP1=0  Tmeas=pv_Tmeas degC  TFIXED=pv_T degC  thermal_mass=100 J/K  initial_temperature=25 degC
  PV_21_3 : ee_lib/Sources/Solar Cell  prm=ee.enum.sources.solar_cell_prm.datasheet  Isc=pv_Isc A  Voc=pv_Voc V  Is=1e-6 A  Is2=0 A  Iph=7.34 A  Ir0=pv_Ir0 W/m^2  ec=pv_n  N2=2  Rs=pv_Rs Ohm  Rp=inf Ohm  N_series=pv_Ngrp  N_parallel=1  TIPH1=pv_TIPH1 1/K  EG=pv_EG eV  TXIS1=pv_TXIS1  TXIS2=3  TRS1=pv_TRS1  TRP1=0  Tmeas=pv_Tmeas degC  TFIXED=pv_T degC  thermal_mass=100 J/K  initial_temperature=25 degC
  PV_22_1 : ee_lib/Sources/Solar Cell  prm=ee.enum.sources.solar_cell_prm.datasheet  Isc=pv_Isc A  Voc=pv_Voc V  Is=1e-6 A  Is2=0 A  Iph=7.34 A  Ir0=pv_Ir0 W/m^2  ec=pv_n  N2=2  Rs=pv_Rs Ohm  Rp=inf Ohm  N_series=pv_Ngrp  N_parallel=1  TIPH1=pv_TIPH1 1/K  EG=pv_EG eV  TXIS1=pv_TXIS1  TXIS2=3  TRS1=pv_TRS1  TRP1=0  Tmeas=pv_Tmeas degC  TFIXED=pv_T degC  thermal_mass=100 J/K  initial_temperature=25 degC
  PV_22_2 : ee_lib/Sources/Solar Cell  prm=ee.enum.sources.solar_cell_prm.datasheet  Isc=pv_Isc A  Voc=pv_Voc V  Is=1e-6 A  Is2=0 A  Iph=7.34 A  Ir0=pv_Ir0 W/m^2  ec=pv_n  N2=2  Rs=pv_Rs Ohm  Rp=inf Ohm  N_series=pv_Ngrp  N_parallel=1  TIPH1=pv_TIPH1 1/K  EG=pv_EG eV  TXIS1=pv_TXIS1  TXIS2=3  TRS1=pv_TRS1  TRP1=0  Tmeas=pv_Tmeas degC  TFIXED=pv_T degC  thermal_mass=100 J/K  initial_temperature=25 degC
  PV_22_3 : ee_lib/Sources/Solar Cell  prm=ee.enum.sources.solar_cell_prm.datasheet  Isc=pv_Isc A  Voc=pv_Voc V  Is=1e-6 A  Is2=0 A  Iph=7.34 A  Ir0=pv_Ir0 W/m^2  ec=pv_n  N2=2  Rs=pv_Rs Ohm  Rp=inf Ohm  N_series=pv_Ngrp  N_parallel=1  TIPH1=pv_TIPH1 1/K  EG=pv_EG eV  TXIS1=pv_TXIS1  TXIS2=3  TRS1=pv_TRS1  TRP1=0  Tmeas=pv_Tmeas degC  TFIXED=pv_T degC  thermal_mass=100 J/K  initial_temperature=25 degC
  PV_23_1 : ee_lib/Sources/Solar Cell  prm=ee.enum.sources.solar_cell_prm.datasheet  Isc=pv_Isc A  Voc=pv_Voc V  Is=1e-6 A  Is2=0 A  Iph=7.34 A  Ir0=pv_Ir0 W/m^2  ec=pv_n  N2=2  Rs=pv_Rs Ohm  Rp=inf Ohm  N_series=pv_Ngrp  N_parallel=1  TIPH1=pv_TIPH1 1/K  EG=pv_EG eV  TXIS1=pv_TXIS1  TXIS2=3  TRS1=pv_TRS1  TRP1=0  Tmeas=pv_Tmeas degC  TFIXED=pv_T degC  thermal_mass=100 J/K  initial_temperature=25 degC
  PV_23_2 : ee_lib/Sources/Solar Cell  prm=ee.enum.sources.solar_cell_prm.datasheet  Isc=pv_Isc A  Voc=pv_Voc V  Is=1e-6 A  Is2=0 A  Iph=7.34 A  Ir0=pv_Ir0 W/m^2  ec=pv_n  N2=2  Rs=pv_Rs Ohm  Rp=inf Ohm  N_series=pv_Ngrp  N_parallel=1  TIPH1=pv_TIPH1 1/K  EG=pv_EG eV  TXIS1=pv_TXIS1  TXIS2=3  TRS1=pv_TRS1  TRP1=0  Tmeas=pv_Tmeas degC  TFIXED=pv_T degC  thermal_mass=100 J/K  initial_temperature=25 degC
  PV_23_3 : ee_lib/Sources/Solar Cell  prm=ee.enum.sources.solar_cell_prm.datasheet  Isc=pv_Isc A  Voc=pv_Voc V  Is=1e-6 A  Is2=0 A  Iph=7.34 A  Ir0=pv_Ir0 W/m^2  ec=pv_n  N2=2  Rs=pv_Rs Ohm  Rp=inf Ohm  N_series=pv_Ngrp  N_parallel=1  TIPH1=pv_TIPH1 1/K  EG=pv_EG eV  TXIS1=pv_TXIS1  TXIS2=3  TRS1=pv_TRS1  TRP1=0  Tmeas=pv_Tmeas degC  TFIXED=pv_T degC  thermal_mass=100 J/K  initial_temperature=25 degC
  PV_24_1 : ee_lib/Sources/Solar Cell  prm=ee.enum.sources.solar_cell_prm.datasheet  Isc=pv_Isc A  Voc=pv_Voc V  Is=1e-6 A  Is2=0 A  Iph=7.34 A  Ir0=pv_Ir0 W/m^2  ec=pv_n  N2=2  Rs=pv_Rs Ohm  Rp=inf Ohm  N_series=pv_Ngrp  N_parallel=1  TIPH1=pv_TIPH1 1/K  EG=pv_EG eV  TXIS1=pv_TXIS1  TXIS2=3  TRS1=pv_TRS1  TRP1=0  Tmeas=pv_Tmeas degC  TFIXED=pv_T degC  thermal_mass=100 J/K  initial_temperature=25 degC
  PV_24_2 : ee_lib/Sources/Solar Cell  prm=ee.enum.sources.solar_cell_prm.datasheet  Isc=pv_Isc A  Voc=pv_Voc V  Is=1e-6 A  Is2=0 A  Iph=7.34 A  Ir0=pv_Ir0 W/m^2  ec=pv_n  N2=2  Rs=pv_Rs Ohm  Rp=inf Ohm  N_series=pv_Ngrp  N_parallel=1  TIPH1=pv_TIPH1 1/K  EG=pv_EG eV  TXIS1=pv_TXIS1  TXIS2=3  TRS1=pv_TRS1  TRP1=0  Tmeas=pv_Tmeas degC  TFIXED=pv_T degC  thermal_mass=100 J/K  initial_temperature=25 degC
  PV_24_3 : ee_lib/Sources/Solar Cell  prm=ee.enum.sources.solar_cell_prm.datasheet  Isc=pv_Isc A  Voc=pv_Voc V  Is=1e-6 A  Is2=0 A  Iph=7.34 A  Ir0=pv_Ir0 W/m^2  ec=pv_n  N2=2  Rs=pv_Rs Ohm  Rp=inf Ohm  N_series=pv_Ngrp  N_parallel=1  TIPH1=pv_TIPH1 1/K  EG=pv_EG eV  TXIS1=pv_TXIS1  TXIS2=3  TRS1=pv_TRS1  TRP1=0  Tmeas=pv_Tmeas degC  TFIXED=pv_T degC  thermal_mass=100 J/K  initial_temperature=25 degC
  PV_31_1 : ee_lib/Sources/Solar Cell  prm=ee.enum.sources.solar_cell_prm.datasheet  Isc=pv_Isc A  Voc=pv_Voc V  Is=1e-6 A  Is2=0 A  Iph=7.34 A  Ir0=pv_Ir0 W/m^2  ec=pv_n  N2=2  Rs=pv_Rs Ohm  Rp=inf Ohm  N_series=pv_Ngrp  N_parallel=1  TIPH1=pv_TIPH1 1/K  EG=pv_EG eV  TXIS1=pv_TXIS1  TXIS2=3  TRS1=pv_TRS1  TRP1=0  Tmeas=pv_Tmeas degC  TFIXED=pv_T degC  thermal_mass=100 J/K  initial_temperature=25 degC
  PV_31_2 : ee_lib/Sources/Solar Cell  prm=ee.enum.sources.solar_cell_prm.datasheet  Isc=pv_Isc A  Voc=pv_Voc V  Is=1e-6 A  Is2=0 A  Iph=7.34 A  Ir0=pv_Ir0 W/m^2  ec=pv_n  N2=2  Rs=pv_Rs Ohm  Rp=inf Ohm  N_series=pv_Ngrp  N_parallel=1  TIPH1=pv_TIPH1 1/K  EG=pv_EG eV  TXIS1=pv_TXIS1  TXIS2=3  TRS1=pv_TRS1  TRP1=0  Tmeas=pv_Tmeas degC  TFIXED=pv_T degC  thermal_mass=100 J/K  initial_temperature=25 degC
  PV_31_3 : ee_lib/Sources/Solar Cell  prm=ee.enum.sources.solar_cell_prm.datasheet  Isc=pv_Isc A  Voc=pv_Voc V  Is=1e-6 A  Is2=0 A  Iph=7.34 A  Ir0=pv_Ir0 W/m^2  ec=pv_n  N2=2  Rs=pv_Rs Ohm  Rp=inf Ohm  N_series=pv_Ngrp  N_parallel=1  TIPH1=pv_TIPH1 1/K  EG=pv_EG eV  TXIS1=pv_TXIS1  TXIS2=3  TRS1=pv_TRS1  TRP1=0  Tmeas=pv_Tmeas degC  TFIXED=pv_T degC  thermal_mass=100 J/K  initial_temperature=25 degC
  PV_32_1 : ee_lib/Sources/Solar Cell  prm=ee.enum.sources.solar_cell_prm.datasheet  Isc=pv_Isc A  Voc=pv_Voc V  Is=1e-6 A  Is2=0 A  Iph=7.34 A  Ir0=pv_Ir0 W/m^2  ec=pv_n  N2=2  Rs=pv_Rs Ohm  Rp=inf Ohm  N_series=pv_Ngrp  N_parallel=1  TIPH1=pv_TIPH1 1/K  EG=pv_EG eV  TXIS1=pv_TXIS1  TXIS2=3  TRS1=pv_TRS1  TRP1=0  Tmeas=pv_Tmeas degC  TFIXED=pv_T degC  thermal_mass=100 J/K  initial_temperature=25 degC
  PV_32_2 : ee_lib/Sources/Solar Cell  prm=ee.enum.sources.solar_cell_prm.datasheet  Isc=pv_Isc A  Voc=pv_Voc V  Is=1e-6 A  Is2=0 A  Iph=7.34 A  Ir0=pv_Ir0 W/m^2  ec=pv_n  N2=2  Rs=pv_Rs Ohm  Rp=inf Ohm  N_series=pv_Ngrp  N_parallel=1  TIPH1=pv_TIPH1 1/K  EG=pv_EG eV  TXIS1=pv_TXIS1  TXIS2=3  TRS1=pv_TRS1  TRP1=0  Tmeas=pv_Tmeas degC  TFIXED=pv_T degC  thermal_mass=100 J/K  initial_temperature=25 degC
  PV_32_3 : ee_lib/Sources/Solar Cell  prm=ee.enum.sources.solar_cell_prm.datasheet  Isc=pv_Isc A  Voc=pv_Voc V  Is=1e-6 A  Is2=0 A  Iph=7.34 A  Ir0=pv_Ir0 W/m^2  ec=pv_n  N2=2  Rs=pv_Rs Ohm  Rp=inf Ohm  N_series=pv_Ngrp  N_parallel=1  TIPH1=pv_TIPH1 1/K  EG=pv_EG eV  TXIS1=pv_TXIS1  TXIS2=3  TRS1=pv_TRS1  TRP1=0  Tmeas=pv_Tmeas degC  TFIXED=pv_T degC  thermal_mass=100 J/K  initial_temperature=25 degC
  PV_33_1 : ee_lib/Sources/Solar Cell  prm=ee.enum.sources.solar_cell_prm.datasheet  Isc=pv_Isc A  Voc=pv_Voc V  Is=1e-6 A  Is2=0 A  Iph=7.34 A  Ir0=pv_Ir0 W/m^2  ec=pv_n  N2=2  Rs=pv_Rs Ohm  Rp=inf Ohm  N_series=pv_Ngrp  N_parallel=1  TIPH1=pv_TIPH1 1/K  EG=pv_EG eV  TXIS1=pv_TXIS1  TXIS2=3  TRS1=pv_TRS1  TRP1=0  Tmeas=pv_Tmeas degC  TFIXED=pv_T degC  thermal_mass=100 J/K  initial_temperature=25 degC
  PV_33_2 : ee_lib/Sources/Solar Cell  prm=ee.enum.sources.solar_cell_prm.datasheet  Isc=pv_Isc A  Voc=pv_Voc V  Is=1e-6 A  Is2=0 A  Iph=7.34 A  Ir0=pv_Ir0 W/m^2  ec=pv_n  N2=2  Rs=pv_Rs Ohm  Rp=inf Ohm  N_series=pv_Ngrp  N_parallel=1  TIPH1=pv_TIPH1 1/K  EG=pv_EG eV  TXIS1=pv_TXIS1  TXIS2=3  TRS1=pv_TRS1  TRP1=0  Tmeas=pv_Tmeas degC  TFIXED=pv_T degC  thermal_mass=100 J/K  initial_temperature=25 degC
  PV_33_3 : ee_lib/Sources/Solar Cell  prm=ee.enum.sources.solar_cell_prm.datasheet  Isc=pv_Isc A  Voc=pv_Voc V  Is=1e-6 A  Is2=0 A  Iph=7.34 A  Ir0=pv_Ir0 W/m^2  ec=pv_n  N2=2  Rs=pv_Rs Ohm  Rp=inf Ohm  N_series=pv_Ngrp  N_parallel=1  TIPH1=pv_TIPH1 1/K  EG=pv_EG eV  TXIS1=pv_TXIS1  TXIS2=3  TRS1=pv_TRS1  TRP1=0  Tmeas=pv_Tmeas degC  TFIXED=pv_T degC  thermal_mass=100 J/K  initial_temperature=25 degC
  PV_34_1 : ee_lib/Sources/Solar Cell  prm=ee.enum.sources.solar_cell_prm.datasheet  Isc=pv_Isc A  Voc=pv_Voc V  Is=1e-6 A  Is2=0 A  Iph=7.34 A  Ir0=pv_Ir0 W/m^2  ec=pv_n  N2=2  Rs=pv_Rs Ohm  Rp=inf Ohm  N_series=pv_Ngrp  N_parallel=1  TIPH1=pv_TIPH1 1/K  EG=pv_EG eV  TXIS1=pv_TXIS1  TXIS2=3  TRS1=pv_TRS1  TRP1=0  Tmeas=pv_Tmeas degC  TFIXED=pv_T degC  thermal_mass=100 J/K  initial_temperature=25 degC
  PV_34_2 : ee_lib/Sources/Solar Cell  prm=ee.enum.sources.solar_cell_prm.datasheet  Isc=pv_Isc A  Voc=pv_Voc V  Is=1e-6 A  Is2=0 A  Iph=7.34 A  Ir0=pv_Ir0 W/m^2  ec=pv_n  N2=2  Rs=pv_Rs Ohm  Rp=inf Ohm  N_series=pv_Ngrp  N_parallel=1  TIPH1=pv_TIPH1 1/K  EG=pv_EG eV  TXIS1=pv_TXIS1  TXIS2=3  TRS1=pv_TRS1  TRP1=0  Tmeas=pv_Tmeas degC  TFIXED=pv_T degC  thermal_mass=100 J/K  initial_temperature=25 degC
  PV_34_3 : ee_lib/Sources/Solar Cell  prm=ee.enum.sources.solar_cell_prm.datasheet  Isc=pv_Isc A  Voc=pv_Voc V  Is=1e-6 A  Is2=0 A  Iph=7.34 A  Ir0=pv_Ir0 W/m^2  ec=pv_n  N2=2  Rs=pv_Rs Ohm  Rp=inf Ohm  N_series=pv_Ngrp  N_parallel=1  TIPH1=pv_TIPH1 1/K  EG=pv_EG eV  TXIS1=pv_TXIS1  TXIS2=3  TRS1=pv_TRS1  TRP1=0  Tmeas=pv_Tmeas degC  TFIXED=pv_T degC  thermal_mass=100 J/K  initial_temperature=25 degC
  PV_41_1 : ee_lib/Sources/Solar Cell  prm=ee.enum.sources.solar_cell_prm.datasheet  Isc=pv_Isc A  Voc=pv_Voc V  Is=1e-6 A  Is2=0 A  Iph=7.34 A  Ir0=pv_Ir0 W/m^2  ec=pv_n  N2=2  Rs=pv_Rs Ohm  Rp=inf Ohm  N_series=pv_Ngrp  N_parallel=1  TIPH1=pv_TIPH1 1/K  EG=pv_EG eV  TXIS1=pv_TXIS1  TXIS2=3  TRS1=pv_TRS1  TRP1=0  Tmeas=pv_Tmeas degC  TFIXED=pv_T degC  thermal_mass=100 J/K  initial_temperature=25 degC
  PV_41_2 : ee_lib/Sources/Solar Cell  prm=ee.enum.sources.solar_cell_prm.datasheet  Isc=pv_Isc A  Voc=pv_Voc V  Is=1e-6 A  Is2=0 A  Iph=7.34 A  Ir0=pv_Ir0 W/m^2  ec=pv_n  N2=2  Rs=pv_Rs Ohm  Rp=inf Ohm  N_series=pv_Ngrp  N_parallel=1  TIPH1=pv_TIPH1 1/K  EG=pv_EG eV  TXIS1=pv_TXIS1  TXIS2=3  TRS1=pv_TRS1  TRP1=0  Tmeas=pv_Tmeas degC  TFIXED=pv_T degC  thermal_mass=100 J/K  initial_temperature=25 degC
  PV_41_3 : ee_lib/Sources/Solar Cell  prm=ee.enum.sources.solar_cell_prm.datasheet  Isc=pv_Isc A  Voc=pv_Voc V  Is=1e-6 A  Is2=0 A  Iph=7.34 A  Ir0=pv_Ir0 W/m^2  ec=pv_n  N2=2  Rs=pv_Rs Ohm  Rp=inf Ohm  N_series=pv_Ngrp  N_parallel=1  TIPH1=pv_TIPH1 1/K  EG=pv_EG eV  TXIS1=pv_TXIS1  TXIS2=3  TRS1=pv_TRS1  TRP1=0  Tmeas=pv_Tmeas degC  TFIXED=pv_T degC  thermal_mass=100 J/K  initial_temperature=25 degC
  PV_42_1 : ee_lib/Sources/Solar Cell  prm=ee.enum.sources.solar_cell_prm.datasheet  Isc=pv_Isc A  Voc=pv_Voc V  Is=1e-6 A  Is2=0 A  Iph=7.34 A  Ir0=pv_Ir0 W/m^2  ec=pv_n  N2=2  Rs=pv_Rs Ohm  Rp=inf Ohm  N_series=pv_Ngrp  N_parallel=1  TIPH1=pv_TIPH1 1/K  EG=pv_EG eV  TXIS1=pv_TXIS1  TXIS2=3  TRS1=pv_TRS1  TRP1=0  Tmeas=pv_Tmeas degC  TFIXED=pv_T degC  thermal_mass=100 J/K  initial_temperature=25 degC
  PV_42_2 : ee_lib/Sources/Solar Cell  prm=ee.enum.sources.solar_cell_prm.datasheet  Isc=pv_Isc A  Voc=pv_Voc V  Is=1e-6 A  Is2=0 A  Iph=7.34 A  Ir0=pv_Ir0 W/m^2  ec=pv_n  N2=2  Rs=pv_Rs Ohm  Rp=inf Ohm  N_series=pv_Ngrp  N_parallel=1  TIPH1=pv_TIPH1 1/K  EG=pv_EG eV  TXIS1=pv_TXIS1  TXIS2=3  TRS1=pv_TRS1  TRP1=0  Tmeas=pv_Tmeas degC  TFIXED=pv_T degC  thermal_mass=100 J/K  initial_temperature=25 degC
  PV_42_3 : ee_lib/Sources/Solar Cell  prm=ee.enum.sources.solar_cell_prm.datasheet  Isc=pv_Isc A  Voc=pv_Voc V  Is=1e-6 A  Is2=0 A  Iph=7.34 A  Ir0=pv_Ir0 W/m^2  ec=pv_n  N2=2  Rs=pv_Rs Ohm  Rp=inf Ohm  N_series=pv_Ngrp  N_parallel=1  TIPH1=pv_TIPH1 1/K  EG=pv_EG eV  TXIS1=pv_TXIS1  TXIS2=3  TRS1=pv_TRS1  TRP1=0  Tmeas=pv_Tmeas degC  TFIXED=pv_T degC  thermal_mass=100 J/K  initial_temperature=25 degC
  PV_43_1 : ee_lib/Sources/Solar Cell  prm=ee.enum.sources.solar_cell_prm.datasheet  Isc=pv_Isc A  Voc=pv_Voc V  Is=1e-6 A  Is2=0 A  Iph=7.34 A  Ir0=pv_Ir0 W/m^2  ec=pv_n  N2=2  Rs=pv_Rs Ohm  Rp=inf Ohm  N_series=pv_Ngrp  N_parallel=1  TIPH1=pv_TIPH1 1/K  EG=pv_EG eV  TXIS1=pv_TXIS1  TXIS2=3  TRS1=pv_TRS1  TRP1=0  Tmeas=pv_Tmeas degC  TFIXED=pv_T degC  thermal_mass=100 J/K  initial_temperature=25 degC
  PV_43_2 : ee_lib/Sources/Solar Cell  prm=ee.enum.sources.solar_cell_prm.datasheet  Isc=pv_Isc A  Voc=pv_Voc V  Is=1e-6 A  Is2=0 A  Iph=7.34 A  Ir0=pv_Ir0 W/m^2  ec=pv_n  N2=2  Rs=pv_Rs Ohm  Rp=inf Ohm  N_series=pv_Ngrp  N_parallel=1  TIPH1=pv_TIPH1 1/K  EG=pv_EG eV  TXIS1=pv_TXIS1  TXIS2=3  TRS1=pv_TRS1  TRP1=0  Tmeas=pv_Tmeas degC  TFIXED=pv_T degC  thermal_mass=100 J/K  initial_temperature=25 degC
  PV_43_3 : ee_lib/Sources/Solar Cell  prm=ee.enum.sources.solar_cell_prm.datasheet  Isc=pv_Isc A  Voc=pv_Voc V  Is=1e-6 A  Is2=0 A  Iph=7.34 A  Ir0=pv_Ir0 W/m^2  ec=pv_n  N2=2  Rs=pv_Rs Ohm  Rp=inf Ohm  N_series=pv_Ngrp  N_parallel=1  TIPH1=pv_TIPH1 1/K  EG=pv_EG eV  TXIS1=pv_TXIS1  TXIS2=3  TRS1=pv_TRS1  TRP1=0  Tmeas=pv_Tmeas degC  TFIXED=pv_T degC  thermal_mass=100 J/K  initial_temperature=25 degC
  PV_44_1 : ee_lib/Sources/Solar Cell  prm=ee.enum.sources.solar_cell_prm.datasheet  Isc=pv_Isc A  Voc=pv_Voc V  Is=1e-6 A  Is2=0 A  Iph=7.34 A  Ir0=pv_Ir0 W/m^2  ec=pv_n  N2=2  Rs=pv_Rs Ohm  Rp=inf Ohm  N_series=pv_Ngrp  N_parallel=1  TIPH1=pv_TIPH1 1/K  EG=pv_EG eV  TXIS1=pv_TXIS1  TXIS2=3  TRS1=pv_TRS1  TRP1=0  Tmeas=pv_Tmeas degC  TFIXED=pv_T degC  thermal_mass=100 J/K  initial_temperature=25 degC
  PV_44_2 : ee_lib/Sources/Solar Cell  prm=ee.enum.sources.solar_cell_prm.datasheet  Isc=pv_Isc A  Voc=pv_Voc V  Is=1e-6 A  Is2=0 A  Iph=7.34 A  Ir0=pv_Ir0 W/m^2  ec=pv_n  N2=2  Rs=pv_Rs Ohm  Rp=inf Ohm  N_series=pv_Ngrp  N_parallel=1  TIPH1=pv_TIPH1 1/K  EG=pv_EG eV  TXIS1=pv_TXIS1  TXIS2=3  TRS1=pv_TRS1  TRP1=0  Tmeas=pv_Tmeas degC  TFIXED=pv_T degC  thermal_mass=100 J/K  initial_temperature=25 degC
  PV_44_3 : ee_lib/Sources/Solar Cell  prm=ee.enum.sources.solar_cell_prm.datasheet  Isc=pv_Isc A  Voc=pv_Voc V  Is=1e-6 A  Is2=0 A  Iph=7.34 A  Ir0=pv_Ir0 W/m^2  ec=pv_n  N2=2  Rs=pv_Rs Ohm  Rp=inf Ohm  N_series=pv_Ngrp  N_parallel=1  TIPH1=pv_TIPH1 1/K  EG=pv_EG eV  TXIS1=pv_TXIS1  TXIS2=3  TRS1=pv_TRS1  TRP1=0  Tmeas=pv_Tmeas degC  TFIXED=pv_T degC  thermal_mass=100 J/K  initial_temperature=25 degC
  + : PMIOPort  Side=Right
  - : PMIOPort  Port=2  Side=Right
  wires:
  G/1 -> Demux/1
  Demux/1 -> G_11_1/1
  Demux/2 -> G_11_2/1
  Demux/3 -> G_11_3/1
  Demux/4 -> G_21_1/1
  Demux/5 -> G_21_2/1
  Demux/6 -> G_21_3/1
  Demux/7 -> G_31_1/1
  Demux/8 -> G_31_2/1
  Demux/9 -> G_31_3/1
  Demux/10 -> G_41_1/1
  Demux/11 -> G_41_2/1
  Demux/12 -> G_41_3/1
  Demux/13 -> G_12_1/1
  Demux/14 -> G_12_2/1
  Demux/15 -> G_12_3/1
  Demux/16 -> G_22_1/1
  Demux/17 -> G_22_2/1
  Demux/18 -> G_22_3/1
  Demux/19 -> G_32_1/1
  Demux/20 -> G_32_2/1
  Demux/21 -> G_32_3/1
  Demux/22 -> G_42_1/1
  Demux/23 -> G_42_2/1
  Demux/24 -> G_42_3/1
  Demux/25 -> G_13_1/1
  Demux/26 -> G_13_2/1
  Demux/27 -> G_13_3/1
  Demux/28 -> G_23_1/1
  Demux/29 -> G_23_2/1
  Demux/30 -> G_23_3/1
  Demux/31 -> G_33_1/1
  Demux/32 -> G_33_2/1
  Demux/33 -> G_33_3/1
  Demux/34 -> G_43_1/1
  Demux/35 -> G_43_2/1
  Demux/36 -> G_43_3/1
  Demux/37 -> G_14_1/1
  Demux/38 -> G_14_2/1
  Demux/39 -> G_14_3/1
  Demux/40 -> G_24_1/1
  Demux/41 -> G_24_2/1
  Demux/42 -> G_24_3/1
  Demux/43 -> G_34_1/1
  Demux/44 -> G_34_2/1
  Demux/45 -> G_34_3/1
  Demux/46 -> G_44_1/1
  Demux/47 -> G_44_2/1
  Demux/48 -> G_44_3/1
  connections:
  G_11_1/RConn1 -- PV_11_1/LConn1
  G_11_2/RConn1 -- PV_11_2/LConn1
  PV_11_2/LConn2 -- D_11_2/RConn1 -- D_11_1/LConn1 -- PV_11_1/RConn1
  G_11_3/RConn1 -- PV_11_3/LConn1
  PV_11_3/LConn2 -- D_11_3/RConn1 -- D_11_2/LConn1 -- PV_11_2/RConn1
  G_21_1/RConn1 -- PV_21_1/LConn1
  PV_21_1/LConn2 -- D_21_1/RConn1 -- D_11_3/LConn1 -- PV_11_3/RConn1
  G_21_2/RConn1 -- PV_21_2/LConn1
  PV_21_2/LConn2 -- D_21_2/RConn1 -- D_21_1/LConn1 -- PV_21_1/RConn1
  G_21_3/RConn1 -- PV_21_3/LConn1
  PV_21_3/LConn2 -- D_21_3/RConn1 -- D_21_2/LConn1 -- PV_21_2/RConn1
  G_31_1/RConn1 -- PV_31_1/LConn1
  PV_31_1/LConn2 -- D_31_1/RConn1 -- D_21_3/LConn1 -- PV_21_3/RConn1
  G_31_2/RConn1 -- PV_31_2/LConn1
  PV_31_2/LConn2 -- D_31_2/RConn1 -- D_31_1/LConn1 -- PV_31_1/RConn1
  G_31_3/RConn1 -- PV_31_3/LConn1
  PV_31_3/LConn2 -- D_31_3/RConn1 -- D_31_2/LConn1 -- PV_31_2/RConn1
  G_41_1/RConn1 -- PV_41_1/LConn1
  PV_41_1/LConn2 -- D_41_1/RConn1 -- D_31_3/LConn1 -- PV_31_3/RConn1
  G_41_2/RConn1 -- PV_41_2/LConn1
  PV_41_2/LConn2 -- D_41_2/RConn1 -- D_41_1/LConn1 -- PV_41_1/RConn1
  G_41_3/RConn1 -- PV_41_3/LConn1
  PV_41_3/RConn1 -- D_41_3/LConn1 -- D_42_3/LConn1 -- PV_42_3/RConn1 -- D_43_3/LConn1 -- PV_43_3/RConn1 -- -/RConn1 -- D_44_3/LConn1 -- PV_44_3/RConn1
  PV_41_3/LConn2 -- D_41_3/RConn1 -- D_41_2/LConn1 -- PV_41_2/RConn1
  G_12_1/RConn1 -- PV_12_1/LConn1
  G_12_2/RConn1 -- PV_12_2/LConn1
  PV_12_2/LConn2 -- D_12_2/RConn1 -- D_12_1/LConn1 -- PV_12_1/RConn1
  G_12_3/RConn1 -- PV_12_3/LConn1
  PV_12_3/LConn2 -- D_12_3/RConn1 -- D_12_2/LConn1 -- PV_12_2/RConn1
  G_22_1/RConn1 -- PV_22_1/LConn1
  PV_22_1/LConn2 -- D_22_1/RConn1 -- D_12_3/LConn1 -- PV_12_3/RConn1
  G_22_2/RConn1 -- PV_22_2/LConn1
  PV_22_2/LConn2 -- D_22_2/RConn1 -- D_22_1/LConn1 -- PV_22_1/RConn1
  G_22_3/RConn1 -- PV_22_3/LConn1
  PV_22_3/LConn2 -- D_22_3/RConn1 -- D_22_2/LConn1 -- PV_22_2/RConn1
  G_32_1/RConn1 -- PV_32_1/LConn1
  PV_32_1/LConn2 -- D_32_1/RConn1 -- D_22_3/LConn1 -- PV_22_3/RConn1
  G_32_2/RConn1 -- PV_32_2/LConn1
  PV_32_2/LConn2 -- D_32_2/RConn1 -- D_32_1/LConn1 -- PV_32_1/RConn1
  G_32_3/RConn1 -- PV_32_3/LConn1
  PV_32_3/LConn2 -- D_32_3/RConn1 -- D_32_2/LConn1 -- PV_32_2/RConn1
  G_42_1/RConn1 -- PV_42_1/LConn1
  PV_42_1/LConn2 -- D_42_1/RConn1 -- D_32_3/LConn1 -- PV_32_3/RConn1
  G_42_2/RConn1 -- PV_42_2/LConn1
  PV_42_2/LConn2 -- D_42_2/RConn1 -- D_42_1/LConn1 -- PV_42_1/RConn1
  G_42_3/RConn1 -- PV_42_3/LConn1
  PV_42_3/LConn2 -- D_42_3/RConn1 -- D_42_2/LConn1 -- PV_42_2/RConn1
  G_13_1/RConn1 -- PV_13_1/LConn1
  G_13_2/RConn1 -- PV_13_2/LConn1
  PV_13_2/LConn2 -- D_13_2/RConn1 -- D_13_1/LConn1 -- PV_13_1/RConn1
  G_13_3/RConn1 -- PV_13_3/LConn1
  PV_13_3/LConn2 -- D_13_3/RConn1 -- D_13_2/LConn1 -- PV_13_2/RConn1
  G_23_1/RConn1 -- PV_23_1/LConn1
  PV_23_1/LConn2 -- D_23_1/RConn1 -- D_13_3/LConn1 -- PV_13_3/RConn1
  G_23_2/RConn1 -- PV_23_2/LConn1
  PV_23_2/LConn2 -- D_23_2/RConn1 -- D_23_1/LConn1 -- PV_23_1/RConn1
  G_23_3/RConn1 -- PV_23_3/LConn1
  PV_23_3/LConn2 -- D_23_3/RConn1 -- D_23_2/LConn1 -- PV_23_2/RConn1
  G_33_1/RConn1 -- PV_33_1/LConn1
  PV_33_1/LConn2 -- D_33_1/RConn1 -- D_23_3/LConn1 -- PV_23_3/RConn1
  G_33_2/RConn1 -- PV_33_2/LConn1
  PV_33_2/LConn2 -- D_33_2/RConn1 -- D_33_1/LConn1 -- PV_33_1/RConn1
  G_33_3/RConn1 -- PV_33_3/LConn1
  PV_33_3/LConn2 -- D_33_3/RConn1 -- D_33_2/LConn1 -- PV_33_2/RConn1
  G_43_1/RConn1 -- PV_43_1/LConn1
  PV_43_1/LConn2 -- D_43_1/RConn1 -- D_33_3/LConn1 -- PV_33_3/RConn1
  G_43_2/RConn1 -- PV_43_2/LConn1
  PV_43_2/LConn2 -- D_43_2/RConn1 -- D_43_1/LConn1 -- PV_43_1/RConn1
  G_43_3/RConn1 -- PV_43_3/LConn1
  PV_43_3/LConn2 -- D_43_3/RConn1 -- D_43_2/LConn1 -- PV_43_2/RConn1
  G_14_1/RConn1 -- PV_14_1/LConn1
  PV_14_1/LConn2 -- D_14_1/RConn1 -- +/RConn1 -- D_11_1/RConn1 -- PV_11_1/LConn2 -- D_12_1/RConn1 -- PV_12_1/LConn2 -- D_13_1/RConn1 -- PV_13_1/LConn2
  G_14_2/RConn1 -- PV_14_2/LConn1
  PV_14_2/LConn2 -- D_14_2/RConn1 -- D_14_1/LConn1 -- PV_14_1/RConn1
  G_14_3/RConn1 -- PV_14_3/LConn1
  PV_14_3/LConn2 -- D_14_3/RConn1 -- D_14_2/LConn1 -- PV_14_2/RConn1
  G_24_1/RConn1 -- PV_24_1/LConn1
  PV_24_1/LConn2 -- D_24_1/RConn1 -- D_14_3/LConn1 -- PV_14_3/RConn1
  G_24_2/RConn1 -- PV_24_2/LConn1
  PV_24_2/LConn2 -- D_24_2/RConn1 -- D_24_1/LConn1 -- PV_24_1/RConn1
  G_24_3/RConn1 -- PV_24_3/LConn1
  PV_24_3/LConn2 -- D_24_3/RConn1 -- D_24_2/LConn1 -- PV_24_2/RConn1
  G_34_1/RConn1 -- PV_34_1/LConn1
  PV_34_1/LConn2 -- D_34_1/RConn1 -- D_24_3/LConn1 -- PV_24_3/RConn1
  G_34_2/RConn1 -- PV_34_2/LConn1
  PV_34_2/LConn2 -- D_34_2/RConn1 -- D_34_1/LConn1 -- PV_34_1/RConn1
  G_34_3/RConn1 -- PV_34_3/LConn1
  PV_34_3/LConn2 -- D_34_3/RConn1 -- D_34_2/LConn1 -- PV_34_2/RConn1
  G_44_1/RConn1 -- PV_44_1/LConn1
  PV_44_1/LConn2 -- D_44_1/RConn1 -- D_34_3/LConn1 -- PV_34_3/RConn1
  G_44_2/RConn1 -- PV_44_2/LConn1
  PV_44_2/LConn2 -- D_44_2/RConn1 -- D_44_1/LConn1 -- PV_44_1/RConn1
  G_44_3/RConn1 -- PV_44_3/LConn1
  PV_44_3/LConn2 -- D_44_3/RConn1 -- D_44_2/LConn1 -- PV_44_2/RConn1
